simulink model "ASM_Traffic_new"  (R2024a)
settings: Solver=ode1  StartTime=SIM.tstart.v  StopTime=SIM.tend.v  FixedStep=SIM.StepSize.v  RelTol=1e-3
PostLoadFcn:
  | if any(exist('dsrtsu_mdlpostloadfcn', 'file') ~= 0), dsrtsu_mdlpostloadfcn('Execute', bdroot); end
  | try, asm_mdl_postloadfcn(bdroot, 'UpdateModel', 3600); catch, disp(lasterr); end,
InitFcn:
  | , if any(exist('rtifpga_mdlclblib', 'file') ~= 0), rtifpga_mdlclblib('Init', bdroot); end,
  | , if any(exist('dsmpb_private', 'file') ~= 0), dsmpb_private('dsmpb_mdlclblib', 'Init', bdroot); end,
undefined symbols (not defined in the file): _to_, a0b2, ASM_BrakeHydraulics_DemoSystems, ASM_VehicleDynamics_DemoSystems, b98103fe8ad365046cd0, BrakeCircuit, CPT, Crankshaft, DiscIntNeverNeededParam, dsmsi, FinalDriveAssembly, MDL, ModeSignals, Pos_BrakePedal_Maneuver, rad, RefSignals, s_to_rpm, SIM, SoftECU, Suspension, Tire, Transmission
libraries: ASM_Traffic_lib x135, simulink x100, ASM_Utils_lib x77, ASM_VehicleDynamics_lib x70, ASM_Environment_lib x22, dsmpblib x20, dsmsilib x15, MDLD_Utils_lib x10, ASM_BrakeHydraulics_lib x3
(part 32 of 63)

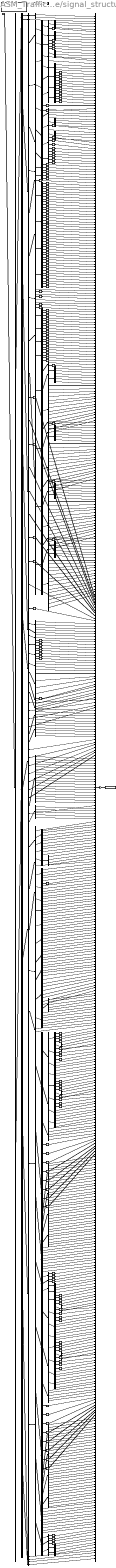
== system ASM_Traffic_new/VehicleDynamics/SignalInterface/ASMSignalInterface/signal_structure ==
  ASMSignalBus : Inport
  Accelerations : BusSelector  OutputSignals=VehicleCoG,Wheels
  ActiveBrakeCylinder : BusSelector  OutputSignals=p[bar],p_max[bar],Enable_p_Brake_Desired[0|1],p_Brake_Desired[bar]
  Aerodynamics : BusSelector  OutputSignals=Forces,Torques,Coefficients
  Angle_FL_Wheel[Toe;Camber][deg] : BusSelector  OutputSignals=Angle_Toe_FL_Wheel_CoorSys_V[deg],Angle_Camber_FL_Wheel_CoorSys_V[deg]
  Angle_FR_Wheel[Toe;Camber][deg] : BusSelector  OutputSignals=Angle_Toe_FR_Wheel_CoorSys_V[deg],Angle_Camber_FR_Wheel_CoorSys_V[deg]
  Angle_Left_Wheel[Alpha;Beta;Gamma][deg] : BusSelector  OutputSignals=Angle_Alpha_Left_Wheel[deg],Angle_Beta_Left_Wheel[deg],Angle_Gamma_Left_Wheel[deg]
  Angle_Left_Wheel[Alpha;Beta;Gamma][deg]1 : BusSelector  OutputSignals=Angle_Alpha_Left_Wheel[deg],Angle_Beta_Left_Wheel[deg],Angle_Gamma_Left_Wheel[deg]
  Angle_RL_Wheel[Toe;Camber][deg] : BusSelector  OutputSignals=Angle_Toe_RL_Wheel_CoorSys_V[deg],Angle_Camber_RL_Wheel_CoorSys_V[deg]
  Angle_RR_Wheel[Toe;Camber][deg] : BusSelector  OutputSignals=Angle_Toe_RR_Wheel_CoorSys_V[deg],Angle_Camber_RR_Wheel_CoorSys_V[deg]
  Angle_Right_Wheel[Alpha;Beta;Gamma][deg] : BusSelector  OutputSignals=Angle_Alpha_Right_Wheel[deg],Angle_Beta_Right_Wheel[deg],Angle_Gamma_Right_Wheel[deg]
  Angle_Right_Wheel[Alpha;Beta;Gamma][deg]1 : BusSelector  OutputSignals=Angle_Alpha_Right_Wheel[deg],Angle_Beta_Right_Wheel[deg],Angle_Gamma_Right_Wheel[deg]
  Angle_Vehicle_CoorSys_E[x;y;z][deg] : BusSelector  OutputSignals=Angle_Roll_Vehicle_CoorSys_E[deg],Angle_Pitch_Vehicle_CoorSys_E[deg],Angle_Yaw_Vehicle_CoorSys_E[deg]
  Angle_Wheel[FL;FR][Toe;Camber][deg] : BusSelector  OutputSignals=Angle_FL_Wheel[Toe;Camber][deg],Angle_FR_Wheel[Toe;Camber][deg]
  Angle_Wheel[RL;RR][Toe;Camber][deg] : BusSelector  OutputSignals=Angle_RL_Wheel[Toe;Camber][deg],Angle_RR_Wheel[Toe;Camber][deg]
  Angular : BusSelector  OutputSignals=w_Vehicle_CoG_dt[x;y;z][rad|s2]
  Angular1 : BusSelector  OutputSignals=w_Vehicle_CoG[x;y;z][deg|s]
  Angular2 : BusSelector  OutputSignals=WheelBodyAngularVelocity,WheelAngularVelocity
  Angular3 : BusSelector  OutputSignals=Angle_Vehicle_CoorSys_E[x;y;z][deg],Angle_V[Alpha;Beta;Gamma][deg],RotationMatrix_V_to_E[3x3],RotationMatrix_V_to_E[1x9],RotationMatrix_V_to_E_T[3x3],RotationMatrix_V_to_E_T[1x9]
  BellValve : BusSelector  OutputSignals=ValveState[1ChamberCon|2AmbientCon|3CloseAll],p_In_BellValve[bar],p_Out_BellValve[bar],T_In_BellValve[degC],m_dot_BellValve[kg|s],Ctrl_BellValve[0_1]
  Brake : BusSelector  OutputSignals=MasterBrakeCylinder,BrakeHydraulics,BrakeDisc,VacuumServo,Manifold
  BrakeCylinderLinear : BusSelector  OutputSignals=p[bar],p_max[bar]
  BrakeCylinderPhysical : BusSelector  OutputSignals=Displ_Piston[mm],F[N],p[bar],p_max[bar]
  BrakeDisc : BusSelector  OutputSignals=Torque,MaximumTorque,Pressure,Const_BrakeDiscFactor
  BrakeHydraulics : BusSelector  OutputSignals=BrakingCircuit,BrakeHydraulicsModel[]
  BrakingCircuit : BusSelector  OutputSignals=Pressure
  BusSelector_1 : BusSelector  OutputSignals=Control,Plant
  Coefficients : BusSelector  OutputSignals=Cw_x[]
  ComplianceAligningTorque : BusSelector  OutputSignals=Displ_x_Wheel_Trq_z_Left[mm],Displ_x_Wheel_Trq_z_Right[mm],Displ_y_Wheel_Trq_z_Left[mm],Displ_y_Wheel_Trq_z_Right[mm],Angle_Alpha_Wheel_Trq_z_Left[deg],Angle_Alpha_Wheel_Trq_z_Right[deg],Angle_Gamma_Wheel_Trq_z_Left[deg],Angle_Gamma_Wheel_Trq_z_Right[deg]
  ComplianceAligningTorque1 : BusSelector  OutputSignals=Displ_x_Wheel_Trq_z_Left[mm],Displ_x_Wheel_Trq_z_Right[mm],Displ_y_Wheel_Trq_z_Left[mm],Displ_y_Wheel_Trq_z_Right[mm],Angle_Alpha_Wheel_Trq_z_Left[deg],Angle_Alpha_Wheel_Trq_z_Right[deg],Angle_Gamma_Wheel_Trq_z_Left[deg],Angle_Gamma_Wheel_Trq_z_Right[deg]
  ComplianceLatForce : BusSelector  OutputSignals=Displ_x_Wheel_F_y_Left[mm],Displ_x_Wheel_F_y_Right[mm],Displ_y_Wheel_F_y_Left[mm],Displ_y_Wheel_F_y_Right[mm],Angle_Alpha_Wheel_F_y_Left[deg],Angle_Alpha_Wheel_F_y_Right[deg],Angle_Gamma_Wheel_F_y_Left[deg],Angle_Gamma_Wheel_F_y_Right[deg]
  ComplianceLatForce1 : BusSelector  OutputSignals=Displ_x_Wheel_F_y_Left[mm],Displ_x_Wheel_F_y_Right[mm],Displ_y_Wheel_F_y_Left[mm],Displ_y_Wheel_F_y_Right[mm],Angle_Alpha_Wheel_F_y_Left[deg],Angle_Alpha_Wheel_F_y_Right[deg],Angle_Gamma_Wheel_F_y_Left[deg],Angle_Gamma_Wheel_F_y_Right[deg]
  ComplianceLongForce : BusSelector  OutputSignals=Displ_x_Wheel_F_x_Left[mm],Displ_x_Wheel_F_x_Right[mm],Displ_y_Wheel_F_x_Left[mm],Displ_y_Wheel_F_x_Right[mm],Angle_Alpha_Wheel_F_x_Left[deg],Angle_Alpha_Wheel_F_x_Right[deg],Angle_Gamma_Wheel_F_x_Left[deg],Angle_Gamma_Wheel_F_x_Right[deg]
  ComplianceLongForce1 : BusSelector  OutputSignals=Displ_x_Wheel_F_x_Left[mm],Displ_x_Wheel_F_x_Right[mm],Displ_y_Wheel_F_x_Left[mm],Displ_y_Wheel_F_x_Right[mm],Angle_Alpha_Wheel_F_x_Left[deg],Angle_Alpha_Wheel_F_x_Right[deg],Angle_Gamma_Wheel_F_x_Left[deg],Angle_Gamma_Wheel_F_x_Right[deg]
  ComplianceLongTorque : BusSelector  OutputSignals=Displ_x_Wheel_Trq_x_Left[mm],Displ_x_Wheel_Trq_x_Right[mm],Displ_y_Wheel_Trq_x_Left[mm],Displ_y_Wheel_Trq_x_Right[mm],Angle_Alpha_Wheel_Trq_x_Left[deg],Angle_Alpha_Wheel_Trq_x_Right[deg],Angle_Gamma_Wheel_Trq_x_Left[deg],Angle_Gamma_Wheel_Trq_x_Right[deg]
  ComplianceLongTorque1 : BusSelector  OutputSignals=Displ_x_Wheel_Trq_x_Left[mm],Displ_x_Wheel_Trq_x_Right[mm],Displ_y_Wheel_Trq_x_Left[mm],Displ_y_Wheel_Trq_x_Right[mm],Angle_Alpha_Wheel_Trq_x_Left[deg],Angle_Alpha_Wheel_Trq_x_Right[deg],Angle_Gamma_Wheel_Trq_x_Left[deg],Angle_Gamma_Wheel_Trq_x_Right[deg]
  Const_BrakeDiscFactor : BusSelector  OutputSignals=Const_BrakeDiscFactor_FL[m3],Const_BrakeDiscFactor_FR[m3],Const_BrakeDiscFactor_RL[m3],Const_BrakeDiscFactor_RR[m3]
  ContactPoint{,1..3} (4 alike) : BusSelector  OutputSignals=r_Tire[m],Pos_CP_CoorSys_E[x;y][m]
  ContentID : Constant  Value=957506836
  Control : BusSelector  OutputSignals=SoftECU_Brake,SoftECU_PowerSteering
  ControllerBellValve : BusSelector  OutputSignals=p_Setpoint[bar],p_MasterBrakeCyl[bar],p_delta[bar],ValveState[1ChamberCon|2AmbientCon],Ctrl_A_BellValve[0_1],F_Pedal[N]
  Damper_Left : BusSelector  OutputSignals=Displ_Damper_Left_dt[m|s],Displ_Damper_Left_dqL[],Displ_Damper_Left_dqR[],Displ_Damper_Left[m]
  Damper_Left1 : BusSelector  OutputSignals=Displ_Damper_Left_dt[m|s],Displ_Damper_Left_dqL[],Displ_Damper_Left_dqR[],Displ_Damper_Left[m]
  Damper_Right : BusSelector  OutputSignals=Displ_Damper_Right_dt[m|s],Displ_Damper_Right_dqL[],Displ_Damper_Right_dqR[],Displ_Damper_Right[m]
  Damper_Right1 : BusSelector  OutputSignals=Displ_Damper_Right_dt[m|s],Displ_Damper_Right_dqL[],Displ_Damper_Right_dqR[],Displ_Damper_Right[m]
  DesiredBrakePressure : BusSelector  OutputSignals=Enable_p_Brake_Desired[0|1],p_Brake_Desired[bar]
  DrivingResistances : BusSelector  OutputSignals=F_Driving_Res[N]
  F_Tire_CoorSys_V[x;y;z][N]{,1..3} (4 alike) : BusSelector  OutputSignals=F_x_Tire_CoorSys_V[N],F_y_Tire_CoorSys_V[N],F_z_Tire_CoorSys_V[N]
  Forces : BusSelector  OutputSignals=F_x_Aero_CoorSys_V[N],F_y_Aero_CoorSys_V[N],F_z_Aero_CoorSys_V[N]
  ForcesAndTorques : BusSelector  OutputSignals=g_F_Steering_SteeringRod[N],Trq_Steering[Nm],Trq_PowerSteering[Nm],TrqSpring_SteeringColumn[Nm],Trq_PowerSteeringDynamics[Nm],TrqSpring_PowerSteeringSystem[Nm]
  Generalized : BusSelector  OutputSignals=v_Vehicle[x;y;z][km|h],w_Vehicle[x;y;z][deg|s],z_Wheel_dt[FL;FR;RL;RR][m|s]
  GeneralizedForcesAndTorques : BusSelector  OutputSignals=g_F_Vehicle[x;y;z][N],g_Trq_Vehicle[x;y;z][Nm],g_F_z_Wheel[FL;FR;RL;RR][N]
  GeneralizedForcesAndTorques1 : BusSelector  OutputSignals=g_FTrq_Tire_Steering[N],g_Trq_FL_Steering[N],g_Trq_FR_Steering[N],g_F_FL_Steering[N],g_F_FR_Steering[N]
  GeneralizedVelocitiesDerivative : BusSelector  OutputSignals=v_Vehicle_dt[x;y;z][m|s2],w_Vehicle_dt[x;y;z][rad|s2],q_Wheel_dt2[q1_Front;q2_Front;q1_Rear;q2_Rear][]
  GravitationalForces : BusSelector  OutputSignals=F_Vehicle_Gravitational[x;y;z][N],F_FL_Gravitational[x;y;z][N],F_FR_Gravitational[x;y;z][N],F_RL_Gravitational[x;y;z][N],F_RR_Gravitational[x;y;z][N]
  GravityAcceleration : BusSelector  OutputSignals=a_Gravity_CoorSys_V[x;y;z][m|s2]
  GyroscopicForces : BusSelector  OutputSignals=F_Vehicle_Gyroscopic[x;y;z][N],F_FL_Gyroscopic[x;y;z][N],F_FR_Gyroscopic[x;y;z][N],F_RL_Gyroscopic[x;y;z][N],F_RR_Gyroscopic[x;y;z][N]
  GyroscopicTorques : BusSelector  OutputSignals=Trq_Vehicle_Gyroscope[x;y;z][Nm],Trq_FL_Gyroscope[x;y;z][Nm],Trq_FR_Gyroscope[x;y;z][Nm],Trq_RL_Gyroscope[x;y;z][Nm],Trq_RR_Gyroscope[x;y;z][Nm]
  InfoBlock : Subsystem
      mask Display: fprintf('Structural changes of the signal bus require an update \nof the ''ASMSignalCollector'' block. \n\nTo start the update process double click the parent block.\n\n WARNING:\n During update this subsystem will be cleared completely')
  Kinematics_Left : BusSelector  OutputSignals=Position_Left,Orientation_Left,Spring_Left,Damper_Left
  Kinematics_Left1 : BusSelector  OutputSignals=Position_Left,Orientation_Left,Spring_Left,Damper_Left
  Kinematics_Right : BusSelector  OutputSignals=Position_Right,Orientation_Right,Spring_Right,Damper_Right
  Kinematics_Right1 : BusSelector  OutputSignals=Position_Right,Orientation_Right,Spring_Right,Damper_Right
  Linear : BusSelector  OutputSignals=a_Vehicle_CoG[x;y;z][m|s2],a_Vehicle_CoG_withG[x;y;z][m|s2]
  Linear1 : BusSelector  OutputSignals=a_FL_Wheel[x;y;z][m|s2],a_FR_Wheel[x;y;z][m|s2],a_RL_Wheel[x;y;z][m|s2],a_RR_Wheel[x;y;z][m|s2]
  Linear2 : BusSelector  OutputSignals=v_Vehicle_CoG[x;y;z][km|h],v_Total_Vehicle[km|h],Angle_SideSlip_Vehicle[deg]
  Linear3 : BusSelector  OutputSignals=WheelBodyVelocity
  Linear4 : BusSelector  OutputSignals=Pos_Vehicle_CoorSys_E[x;y;z][m],Pos_Vehicle_CoorSys_E[m],s_Vehicle[m]
  Linear5 : BusSelector  OutputSignals=Pos_FL_Wheels_CoorSys_E[x;y;z][m],Pos_FR_Wheels_CoorSys_E[x;y;z][m],Pos_RL_Wheels_CoorSys_E[x;y;z][m],Pos_RR_Wheels_CoorSys_E[x;y;z][m]
  MDLD_DATA_CAPTURE : MDLD_Utils_lib/ModelDeskPlotInterface/DataCapture_Sfcn/MDLD_DATA_CAPTURE  inputPortWidth=976  measurementSignals=[0 0 0 0 0 0 0 0 0 0 0 0 0 0 0 0 0 0 0 0 0 0 0 0 0 0 0 0 0 0 0 0 0 0 0 0 0 0 0 0 0 0 0 0 0 0 0 0 0 0 0 0 0 0 0 0 0 0 0 0 0 0 0 0 0 0 0 0 0 0 0 0 0 0 0 0 0 0 0 0 0 0 0 0 0 0 0 0 0 0 0 0 0 0 0 0 0 0 0 0 0 0 0 0 0 0 0 0 0 0 0 0 0 0 0 0 0 0 0 0 0 0 0 0 0 0 0 0 0 0 0 0 0 0 0 0 0 0 0 0 0 0 0 0 0 0 0 0 0 0 0 0 0 0 0 0 0 0 0 0 0 0 0 0 0 0 0 0 0 0 0 0 0 0 0 0 0 0 0 0 0 0 0 0 0 0 0 0 0 0 0 0 0 0 0 0 0 0 0 0 0 0 0 0 0 0 0 0 0 0 0 0 0 0 0 0 0 0 0 0 0 0 0 0 0 0 0 0 0 0 0 0 0 0 0 0 0 0 0 0 0 0 0 0 0 0 0 0 0 0 0 0 0 0 0 0 0 0 0 0 0 0 0 0 0 0 0 0 0 0 0 0 0 0 0 0 0 0 0 0 0 0 0 0 0 0 0 0 0 0 0 0 0 0 0 0 0 0 0 0 0 0 0 0 0 0 0 0 0 0 0 0 0 0 0 0 0 0 0 0 0 0 0 0 0 0 0 0 0 0 0 0 0 0 0 0 0 0 0 0 0 0 0 0 0 0 0 0 0 0 0 0 0 0 0 0 0 0 0 0 0 0 0 0 0 0 0 0 0 0 0 0 0 0 0 0 0 0 0 0 0 0 0 0 0 0 0 0 0 0 0 0 0 0 0 0 0 0 0 0 0 0 0 0 0 0 0 0 0 0 0 0 0 0 0 0 0 0 0 0 0 0 0 0 0 0 0 0 0 0 0 0 0 0 0 0 0 0 0 0 0 0 0 0 0 0 0 0 0 0 0 0 0 0 0 0 0 0 0 0 0 0 0 0 0 0 0 0 0 0 0 0 0 0 0 0 0 0 0 0 0 0 0 0 0 0 0 0 0 0 0 0 0 0 0 0 0 0 0 0 0 0 0 0 0 0 0 0 0 0 0 0 0 0 0 0 0 0 0 0 0 0 0 0 0 0 0 0 0 0 0 0 0 0 0 0 0 0 0 0 0 0 0 0 0 0 0 0 0 0 0 0 0 0 0 0 0 0 0 0 0 0 0 0 0 0 0 0 0 0 0 0 0 0 0 0 0 0 0 0 0 0 0 0 0 0 0 0 0 0 0 0 0 0 0 0 0 0 0 0 0 0 0 0 0 0 0 0 0 0 0 0 0 0 0 0 0 0 0 0 0 0 0 0 0 0 0 0 0 0 0 0 0 0 0 0 0 0 0 0 0 0 0 0 0 0 0 0 0 0 0 0 0 0 0 0 0 0 0 0 0 0 0 0 0 0 0 0 0 0 0 0 0 0 0 0 0 0 0 0 0 0 0 0 0 0 0 0 0 0 0 0 0 0 0 0 0 0 0 0 0 0 0 0 0 0 0 0 0 0 0 0 0 0 0 0 0 0 0 0 0 0 0 0 0 0 0 0 0 0 0 0 0 0 0 0 0 0 0 0 0 0 0 0 0 0 0 0 0 0 0 0 0 0 0 0 0 0 0 0 0 0 0 0 0 0 0 0 0 0 0 0 0 0 0 0 0 0 0 0 0 0 0 0 0 0 0 0 0 0 0 0 0 0 0 0 0 0 0 0 0 0 0 0 0 0 0 0 0 0 0 0 0 0 0 0 0 0 0 0 0 0 0 0 0 0 0 0 0 0 0 0 0 0 0 0 0 0 0 0 0 0 0 0 0 0 0 0 0 0 0 0 0 0 0 0 0 0 0 0 0 0 0 0 0 0 0 0 0 0 0 0 0 0 0 0 0 0 0 0 0 0 0 0 0 0 0 0 0 0 0 0 0 0 0 0 0 0 0 0 0 0 0 0 0 0 0 0 0 0 0 0 0 0 0 0 0 0 0 0 0 0 0 0 0 0 0 0 0 0 0 0 0 0 0 0 0 0 0 0 0 0 0 0 0 0 0 0 0 0 0 0 0 0 0 0 0 0 0 0 0 0 0 0 0 0 0 0 0 0 0 0 0 0 0 0]  downsampling=1  samplingPeriod=SIM.StepSize.v  uuid=0  ASMProperties=struct('Name','mdld_data_capture','Version','1.0','Library','mdld_utils_lib')  startTriggerDelay=0  startTriggerLogic=0  startTriggerCount=0  startTriggerConditions=[0,0,0,0,0,0,0,0,0]  stopTriggerDelay=0  stopTriggerLogic=0  stopTriggerCount=0  stopTriggerConditions=[0,0,0,0,0,0,0,0,0]  ContentID_RefStruct=957506836
  Manifold : BusSelector  OutputSignals=Pos_AccPedal[%],p_Manifold[bar]
  ManifoldValve : BusSelector  OutputSignals=p_In_MainfoldValve[bar],p_Out_MainfoldValve[bar],T_In_MainfoldValve[degC],m_dot_ManifoldValve[kg|s],m_dot_Out_ManifoldValve[kg|s],m_dot_In_ManifoldValve[kg|s]
  MassForcesAndTorques : BusSelector  OutputSignals=GravitationalForces,GyroscopicForces,GyroscopicTorques,ResidualAccelerations
  MasterBrakeCylinder : BusSelector  OutputSignals=Sw_MasterBrakeCylinder_Mode[1linear|2physical|3Booster|4BrakeByWire],ActiveBrakeCylinder,BrakeCylinderLinear,BrakeCylinderPhysical
  MaximumTorque : BusSelector  OutputSignals=Trq_Max_Brake[Nm],Trq_Max_Brake[FL;FR;RL;RR][Nm],Trq_FL_max_Brake[Nm],Trq_FR_max_Brake[Nm],Trq_RL_max_Brake[Nm],Trq_RR_max_Brake[Nm]
  Orientation_Left : BusSelector  OutputSignals=Angle_Left_Wheel[Alpha;Beta;Gamma][deg],w_Rel_Left_Wheel_dqL_dt[x;y;z][rad|m],w_Rel_Left_Wheel_dqR_dt[x;y;z][rad|m],w_Rel_Left_Wheel_dDispl_SteeringRod_dt[x;y;z][rad|m],UnitVec_y_Wheel_Left_CoorSys_V[x;y;z]
  Orientation_Left1 : BusSelector  OutputSignals=Angle_Left_Wheel[Alpha;Beta;Gamma][deg],w_Rel_Left_Wheel_dqL_dt[x;y;z][rad|m],w_Rel_Left_Wheel_dqR_dt[x;y;z][rad|m],w_Rel_Left_Wheel_dDispl_SteeringRod_dt[x;y;z][rad|m],UnitVec_y_Wheel_Left_CoorSys_V[x;y;z]
  Orientation_Right : BusSelector  OutputSignals=Angle_Right_Wheel[Alpha;Beta;Gamma][deg],w_Rel_Right_Wheel_dqL_dt[x;y;z][rad|m],w_Rel_Right_Wheel_dqR_dt[x;y;z][rad|m],w_Rel_Right_Wheel_dDispl_SteeringRod_dt[x;y;z][rad|m],UnitVec_y_Wheel_Right_CoorSys_V[x;y;z]
  Orientation_Right1 : BusSelector  OutputSignals=Angle_Right_Wheel[Alpha;Beta;Gamma][deg],w_Rel_Right_Wheel_dqL_dt[x;y;z][rad|m],w_Rel_Right_Wheel_dqR_dt[x;y;z][rad|m],w_Rel_Right_Wheel_dDispl_SteeringRod_dt[x;y;z][rad|m],UnitVec_y_Wheel_Right_CoorSys_V[x;y;z]
  OutputPoint : BusSelector  OutputSignals=F_OutputPoint[N],p_OutputPoint[bar],Pos_BrakePedal_OutputPoint[%],F_Max_Pedal[N],p_Max_Booster[bar]
  Plant : BusSelector  OutputSignals=VehicleMovement,Tire,Aerodynamics,Wheel,Steering,Brake,Suspension,SteeringRod_Back_Calc,DrivingResistances
  Pos_Vehicle_CoorSys_E[x;y;z][m] : BusSelector  OutputSignals=Pos_x_Vehicle_CoorSys_E[m],Pos_y_Vehicle_CoorSys_E[m],Pos_z_Vehicle_CoorSys_E[m]
  Pos_Wheel[FL;FR][x;y;z][m] : BusSelector  OutputSignals=Pos_FL_Wheel[x;y;z][m],Pos_FR_Wheel[x;y;z][m]
  Pos_Wheel[RL;RR][x;y;z][m] : BusSelector  OutputSignals=Pos_RL_Wheel[x;y;z][m],Pos_RR_Wheel[x;y;z][m]
  Position_Left : BusSelector  OutputSignals=Pos_Left_Wheel[x;y;z][m],Pos_Left_Wheel_dqL[x;y;z][],Pos_Left_Wheel_dqR[x;y;z][],Pos_Left_Wheel_dDispl_SteeringRod[x;y;z][]
  Position_Left1 : BusSelector  OutputSignals=Pos_Left_Wheel[x;y;z][m],Pos_Left_Wheel_dqL[x;y;z][],Pos_Left_Wheel_dqR[x;y;z][],Pos_Left_Wheel_dDispl_SteeringRod[x;y;z][]
  Position_Right : BusSelector  OutputSignals=Pos_Right_Wheel[x;y;z][m],Pos_Right_Wheel_dqL[x;y;z][],Pos_Right_Wheel_dqR[x;y;z][],Pos_Right_Wheel_dDispl_SteeringRod[x;y;z][]
  Position_Right1 : BusSelector  OutputSignals=Pos_Right_Wheel[x;y;z][m],Pos_Right_Wheel_dqL[x;y;z][],Pos_Right_Wheel_dqR[x;y;z][],Pos_Right_Wheel_dDispl_SteeringRod[x;y;z][]
  Positions : BusSelector  OutputSignals=Vehicle,Wheels
  Pressure : BusSelector  OutputSignals=p_FL_Brake[bar],p_FR_Brake[bar],p_RL_Brake[bar],p_RR_Brake[bar]
  Pressure1 : BusSelector  OutputSignals=p_FL_Brake[bar],p_FR_Brake[bar],p_RL_Brake[bar],p_RR_Brake[bar]
  PushRod : BusSelector  OutputSignals=F_Pedal[N],F_Spring[N],F_RearChamber[N],F_VacuumChamber[N],F_PushRod[N],x[m],V_delta[m3],A_Diaphragm[m2],OutputPoint
  RearChamber : BusSelector  OutputSignals=m_dot_In_RearChamber[kg|s],m_dot_Out_RearChamber[kg|s],T_RearChamber[degC],p_RearChamber[bar],V_RearChamber[m3]
  RelativePositionFront : BusSelector  OutputSignals=Pos_Wheel[FL;FR][x;y;z][m],UnitVec_y_Wheel_CoorSys_V[FL;FR][x;y;z],Angle_Wheel[FL;FR][Toe;Camber][deg]
  RelativePositionRear : BusSelector  OutputSignals=Pos_Wheel[RL;RR][x;y;z][m],UnitVec_y_Wheel_CoorSys_V[RL;RR][x;y;z],Angle_Wheel[RL;RR][Toe;Camber][deg]
  Reshape_{7,11..14,23..36,44,49..104,106,108,111..132,134,156,178,200,221,223,227..228,230,238..245,254,327,384..387,391..394,402..405,409..412,425..432,475..478,483..486,490..493,501..504,508..511,524..531,574..577} (175 alike) : Reshape
  ResidualAccelerations : BusSelector  OutputSignals=a_Vehicle_CoG_Residual[x;y;z][m|s2],a_FL_Residual[x;y;z][m|s2],a_FR_Residual[x;y;z][m|s2],a_RL_Residual[x;y;z][m|s2],a_RR_Residual[x;y;z][m|s2]
  RotationAngle : BusSelector  OutputSignals=Angle_Rot_FL_Wheel[deg],Angle_Rot_FR_Wheel[deg],Angle_Rot_RL_Wheel[deg],Angle_Rot_RR_Wheel[deg]
  Sensor1 : BusSelector  OutputSignals=a_Angular_Sensor1_CoorSys_V[x;y;z][rad|s2],a_Total_Sensor1_CoorSys_V[x;y;z][m|s2],a_Sensor1_CoorSys_V[x;y;z][m|s2],v_Sensor1_CoorSys_V[x;y;z][m|s],w_Sensor1_CoorSys_V[x;y;z][rad|s],a_Angular_Sensor1_CoorSys_VH[x;y;z][rad|s2],a_Total_Sensor1_CoorSys_VH[x;y;z][m|s2],a_Sensor1_CoorSys_VH[x;y;z][m|s2],v_Sensor1_CoorSys_VH[x;y;z][m|s],w_Sensor1_CoorSys_VH[x;y;z][rad|s]
  Sensor2 : BusSelector  OutputSignals=a_Angular_Sensor2_CoorSys_V[x;y;z][rad|s2],a_Total_Sensor2_CoorSys_V[x;y;z][m|s2],a_Sensor2_CoorSys_V[x;y;z][m|s2],v_Sensor2_CoorSys_V[x;y;z][m|s],w_Sensor2_CoorSys_V[x;y;z][rad|s],a_Angular_Sensor2_CoorSys_VH[x;y;z][rad|s2],a_Total_Sensor2_CoorSys_VH[x;y;z][m|s2],a_Sensor2_CoorSys_VH[x;y;z][m|s2],v_Sensor2_CoorSys_VH[x;y;z][m|s],w_Sensor2_CoorSys_VH[x;y;z][rad|s]
  Sensor3 : BusSelector  OutputSignals=a_Angular_Sensor3_CoorSys_V[x;y;z][rad|s2],a_Total_Sensor3_CoorSys_V[x;y;z][m|s2],a_Sensor3_CoorSys_V[x;y;z][m|s2],v_Sensor3_CoorSys_V[x;y;z][m|s],w_Sensor3_CoorSys_V[x;y;z][rad|s],a_Angular_Sensor3_CoorSys_VH[x;y;z][rad|s2],a_Total_Sensor3_CoorSys_VH[x;y;z][m|s2],a_Sensor3_CoorSys_VH[x;y;z][m|s2],v_Sensor3_CoorSys_VH[x;y;z][m|s],w_Sensor3_CoorSys_VH[x;y;z][rad|s]
  Sensor4 : BusSelector  OutputSignals=a_Angular_Sensor4_CoorSys_V[x;y;z][rad|s2],a_Total_Sensor4_CoorSys_V[x;y;z][m|s2],a_Sensor4_CoorSys_V[x;y;z][m|s2],v_Sensor4_CoorSys_V[x;y;z][m|s],w_Sensor4_CoorSys_V[x;y;z][rad|s],a_Angular_Sensor4_CoorSys_VH[x;y;z][rad|s2],a_Total_Sensor4_CoorSys_VH[x;y;z][m|s2],a_Sensor4_CoorSys_VH[x;y;z][m|s2],v_Sensor4_CoorSys_VH[x;y;z][m|s],w_Sensor4_CoorSys_VH[x;y;z][rad|s]
  SensorMotion : BusSelector  OutputSignals=Sensor1,Sensor2,Sensor3,Sensor4
  ShaftsTorques_CoorSys_V : BusSelector  OutputSignals=Trq_Shaft_FL_CoorSys_V[x;y;z][Nm],Trq_Shaft_FR_CoorSys_V[x;y;z][Nm],Trq_Shaft_RL_CoorSys_V[x;y;z][Nm],Trq_Shaft_RR_CoorSys_V[x;y;z][Nm]
  SignalFilter : Mux  Inputs=585
  SignalFilterGain : Gain
  SoftECU_Brake : BusSelector  OutputSignals=DesiredBrakePressure
  SoftECU_PowerSteering : BusSelector  OutputSignals=Trq_PowerSteering[Nm]
  Spring_Left : BusSelector  OutputSignals=Displ_Spring_Left[m],Displ_Spring_Left_dqL[],Displ_Spring_Left_dqR[]
  Spring_Left1 : BusSelector  OutputSignals=Displ_Spring_Left[m],Displ_Spring_Left_dqL[],Displ_Spring_Left_dqR[]
  Spring_Right : BusSelector  OutputSignals=Displ_Spring_Right[m],Displ_Spring_Right_dqL[],Displ_Spring_Right_dqR[]
  Spring_Right1 : BusSelector  OutputSignals=Displ_Spring_Right[m],Displ_Spring_Right_dqL[],Displ_Spring_Right_dqR[]
  Stabilizer : BusSelector  OutputSignals=Displ_Stabilizer[m],Displ_Stabilizer_Left[m],Displ_Stabilizer_Right[m],Displ_Stabilizer_dqL[],Displ_Stabilizer_dqR[]
  Stabilizer1 : BusSelector  OutputSignals=Displ_Stabilizer[m],Displ_Stabilizer_Left[m],Displ_Stabilizer_Right[m],Displ_Stabilizer_dqL[],Displ_Stabilizer_dqR[]
  StatesSteeringSystem : BusSelector  OutputSignals=Angle_EPSSystem[deg],Angle_EPSSystem_dt[deg|s],Angle_LowerSteeringColumn[deg],Angle_LowerSteeringColumn_dt[deg|s],Angle_UpperSteeringColumn[deg],Angle_UpperSteeringColumn_dt[deg|s],Angle_SteeringWheel[deg],Angle_SteeringWheel_dt[deg|s],Displ_Steering[m],Displ_Steering_dt[m|s],Displ_SteeringRod_dt2[m|s2],Angle_SteeringGear[deg],Angle_SteeringGear_dt[deg|s],Angle_EPSPinion[rad],Angle_EPSPinion_dt[rad|s],i_Steering[rad|m],FrictionForce_SteeringRod[N],i_Steering_Wheel2Rod[rad|m]
  Steering : BusSelector  OutputSignals=Displ_Steering[m],Displ_Steering_dt[m|s],Displ_SteeringRod_dt2[m|s2],m_Steering[kg],ForcesAndTorques,GeneralizedForcesAndTorques,i_Steering[rad|m],i_Steering_Mean[],Angle_SteeringGear[deg],Angle_SteeringWheel[deg],Angle_SteeringGear_dt[deg|s],Angle_SteeringWheel_dt[deg|s],Const_Stiffness_SteeringColumn[Nm|rad],StatesSteeringSystem,FrictionTrq_SteeringSystem[Nm],SteeringWheelTorque
  SteeringRod_Back_Calc : BusSelector  OutputSignals=Sw_Backward_SteeringRod_Calc[0Off|1On],Displ_SteeringRod[m],Displ_SteeringRod_dt[m|s]
  SteeringWheelTorque : BusSelector  OutputSignals=TrqSensor_Steering[Nm],Trq_Driver[Nm],g_Trq_SteeringWheel[Nm],TrqFriction_SteeringWheel[Nm],Trq_SteeringWheel[Nm]
  Suspension : BusSelector  OutputSignals=SuspensionFront,SuspensionRear
  SuspensionComplianceFront : BusSelector  OutputSignals=Angle_Comp_FR_Wheel_dt[x;y;z][rad|s],Angle_Comp_FL_Wheel_dt[x;y;z][rad|s],Angle_Comp_FR_Wheel[x;y;z][rad],Angle_Comp_FL_Wheel[x;y;z][rad],Displ_Comp_FR_Wheel_dt[x;y;z][m|s],Displ_Comp_FL_Wheel_dt[x;y;z][m|s],Displ_Comp_FR_Wheel[x;y;z][m],Displ_Comp_FL_Wheel[x;y;z][m],ComplianceLongForce,ComplianceLatForce,ComplianceAligningTorque,ComplianceLongTorque
  SuspensionComplianceRear : BusSelector  OutputSignals=Angle_Comp_RR_Wheel_dt[x;y;z][rad|s],Angle_Comp_RL_Wheel_dt[x;y;z][rad|s],Angle_Comp_RR_Wheel[x;y;z][rad],Angle_Comp_RL_Wheel[x;y;z][rad],Displ_Comp_RR_Wheel_dt[x;y;z][m|s],Displ_Comp_RL_Wheel_dt[x;y;z][m|s],Displ_Comp_RR_Wheel[x;y;z][m],Displ_Comp_RL_Wheel[x;y;z][m],ComplianceLongForce,ComplianceLatForce,ComplianceAligningTorque,ComplianceLongTorque
  SuspensionForcesFront : BusSelector  OutputSignals=F_FL_Spring[N],F_FL_Spring_dDispl_FL_Spring[N|m],F_FL_Damper[N],F_FL_Damper_dDispl_FL_Damper_dt[N|(m|s)],F_Stabilizer[N],F_Stabilizer_dDispl_Stabilizer[N|m],F_FR_Spring[N],F_FR_Spring_dDispl_FR_Spring[N|m],F_FR_Damper[N],F_FR_Damper_dDispl_FR_Damper_dt[N|(m|s)]
  SuspensionForcesRear : BusSelector  OutputSignals=F_RL_Spring[N],F_RL_Spring_dDispl_RL_Spring[N|m],F_RL_Damper[N],F_RL_Damper_dDispl_RL_Damper_dt[N|(m|s)],F_Stabilizer[N],F_Stabilizer_dDispl_Stabilizer[N|m],F_RR_Spring[N],F_RR_Spring_dDispl_RR_Spring[N|m],F_RR_Damper[N],F_RR_Damper_dDispl_RR_Damper_dt[N|(m|s)]
  SuspensionFront : BusSelector  OutputSignals=SuspensionKinematicsFront,SuspensionComplianceFront,SuspensionForcesFront,RelativePositionFront
  SuspensionKinematicsFront : BusSelector  OutputSignals=Kinematics_Left,Kinematics_Right,Stabilizer
  SuspensionKinematicsRear : BusSelector  OutputSignals=Kinematics_Left,Kinematics_Right,Stabilizer
  SuspensionRear : BusSelector  OutputSignals=SuspensionKinematicsRear,SuspensionComplianceRear,SuspensionForcesRear,RelativePositionRear
  Terminator : Terminator
  Tire : BusSelector  OutputSignals=Tire_allSignals,r_Dyn_Tire[FL;FR;RL;RR][m],r_Dyn_Tire_Mean[m],Coef_RollingRes[FL;FR;RL;RR][],Coef_RollingRes_Mean[],CorneringStiffness_Tire_Front[N|rad],CorneringStiffness_Tire_Rear[N|rad],CorneringStiffness[FL;FR;RL;RR][N|rad],Const_r_unloaded_Tire[FL;FR;RL;RR][m],Const_r_unloaded_Tire_Mean[m],Slip_x_Wheel[]
  Tire{1..4} (4 alike) : BusSelector  OutputSignals=v_Circumf_Dyn_Wheel[km|h],Slip_x[],Slip_y[],r_Dyn_Tire[m],CorneringStiffness[N|rad],Coef_RollingRes[],Trq_x_CoorSys_CP[Nm],Trq_y_CoorSys_W[Nm],Trq_z_CoorSys_CP[Nm],F_x_Dyn_Tire_CoorSys_CP[N],F_y_Dyn_Tire_CoorSys_CP[N],F_z_Dyn_Tire_CoorSys_CP[N],Const_r_unloaded_Tire[m],Const_Stiffness_z_Tire[N|m]
  TireForcesAndTorques{,1..3} (4 alike) : BusSelector  OutputSignals=F_Tire_CoorSys_V[x;y;z][N],Trq_Tire_CoorSys_V[x;y;z][Nm]
  TireWheelTorques : BusSelector  OutputSignals=Trq_Tire_Wheel_FL[Nm],Trq_Tire_Wheel_FR[Nm],Trq_Tire_Wheel_RL[Nm],Trq_Tire_Wheel_RR[Nm]
  Tire_FL : BusSelector  OutputSignals=ContactPoint,TireForcesAndTorques,Tire
  Tire_FR : BusSelector  OutputSignals=ContactPoint,TireForcesAndTorques,Tire
  Tire_RL : BusSelector  OutputSignals=ContactPoint,TireForcesAndTorques,Tire
  Tire_RR : BusSelector  OutputSignals=ContactPoint,TireForcesAndTorques,Tire
  Tire_allSignals : BusSelector  OutputSignals=Tire_FL,Tire_FR,Tire_RL,Tire_RR
  Torque : BusSelector  OutputSignals=Trq_FL_Brake[Nm],Trq_FR_Brake[Nm],Trq_RL_Brake[Nm],Trq_RR_Brake[Nm]
  Torques : BusSelector  OutputSignals=Trq_x_Aero_CoorSys_V[Nm],Trq_y_Aero_CoorSys_V[Nm],Trq_z_Aero_CoorSys_V[Nm]
  Trq_Tire_CoorSys_V[x;y;z][Nm]{,1..3} (4 alike) : BusSelector  OutputSignals=Trq_x_Tire_CoorSys_V[Nm],Trq_y_Tire_CoorSys_V[Nm],Trq_z_Tire_CoorSys_V[Nm]
  UnitVec_y_Wheel_CoorSys_V[FL;FR][x;y;z] : BusSelector  OutputSignals=UnitVec_y_FL_Wheel_CoorSys_V[x;y;z],UnitVec_y_FR_Wheel_CoorSys_V[x;y;z]
  UnitVec_y_Wheel_CoorSys_V[RL;RR][x;y;z] : BusSelector  OutputSignals=UnitVec_y_RL_Wheel_CoorSys_V[x;y;z],UnitVec_y_RR_Wheel_CoorSys_V[x;y;z]
  VacuumChamber : BusSelector  OutputSignals=m_dot_In_1_VacuumChamber[kg|s],m_dot_In_2_VacuumChamber[kg|s],m_dot_Out_2_VacuumChamber[kg|s],T_VacuumChamber[degC],p_VacuumChamber[bar],V_VacuumChamber[m3]
  VacuumServo : BusSelector  OutputSignals=ManifoldValve,VacuumChamber,BellValve,RearChamber,PushRod,ControllerBellValve
  Vehicle : BusSelector  OutputSignals=Linear,Angular
  Vehicle1 : BusSelector  OutputSignals=Linear,Angular
  VehicleCoG : BusSelector  OutputSignals=Linear,Angular
  VehicleEquationOfMotion : BusSelector  OutputSignals=GeneralizedForcesAndTorques,GeneralizedVelocitiesDerivative
  VehicleMassAndAdditionalLoads : BusSelector  OutputSignals=m_TotalVehicle[kg],PosVec_CoG_TotalVehicle[x;y;z][m],Pos_x_CoG_Vehicle_Total[m],Inertia_Tensor_TotalVehicle[3x3][kgm2],Inertia_z_Vehicle_Total[kgm2],m_TotalV1[kg],PosVec_CoG_TotalV1[x;y;z][m],Inertia_Tensor_TotalV1[3x3][kgm2]
  VehicleMovement : BusSelector  OutputSignals=Accelerations,Velocities,Positions,VehicleEquationOfMotion,GravityAcceleration,SensorMotion,VehicleMassAndAdditionalLoads,MassForcesAndTorques
  Velocities : BusSelector  OutputSignals=Vehicle,Wheels,Generalized
  Wheel : BusSelector  OutputSignals=WheelSpeed_CoorSys_V,ShaftsTorques_CoorSys_V,TireWheelTorques,WheelSpeed,WheelSpeed2,RotationAngle
  WheelAngularVelocity : BusSelector  OutputSignals=w_FL_Abs_Wheel[x;y;z][rad|s],w_FR_Abs_Wheel[x;y;z][rad|s],w_RL_Abs_Wheel[x;y;z][rad|s],w_RR_Abs_Wheel[x;y;z][rad|s]
  WheelBodyAngularVelocity : BusSelector  OutputSignals=w_FL_Abs_WheelBody[x;y;z][rad|s],w_FR_Abs_WheelBody[x;y;z][rad|s],w_RL_Abs_WheelBody[x;y;z][rad|s],w_RR_Abs_WheelBody[x;y;z][rad|s]
  WheelBodyVelocity : BusSelector  OutputSignals=v_FL_Abs_WheelBody[x;y;z][km|h],v_FR_Abs_WheelBody[x;y;z][km|h],v_RL_Abs_WheelBody[x;y;z][km|h],v_RR_Abs_WheelBody[x;y;z][km|h]
  WheelSpeed : BusSelector  OutputSignals=omega_FL_Wheel[rad|s],omega_FR_Wheel[rad|s],omega_RL_Wheel[rad|s],omega_RR_Wheel[rad|s]
  WheelSpeed2 : BusSelector  OutputSignals=omega_Wheel[FL;FR;RL;RR][rad|s],omega_Mean_Wheel[rad|s]
  WheelSpeed_CoorSys_V : BusSelector  OutputSignals=w_Wheel_FL_CoorSys_V[x;y;z][rad|s],w_Wheel_FR_CoorSys_V[x;y;z][rad|s],w_Wheel_RL_CoorSys_V[x;y;z][rad|s],w_Wheel_RR_CoorSys_V[x;y;z][rad|s]
  Wheels : BusSelector  OutputSignals=Linear
  Wheels1 : BusSelector  OutputSignals=Linear,Angular
  Wheels2 : BusSelector  OutputSignals=Linear
  a_Vehicle_CoG[x;y;z][m|s2] : BusSelector  OutputSignals=a_x_Vehicle_CoG[m|s2],a_y_Vehicle_CoG[m|s2],a_z_Vehicle_CoG[m|s2]
  v_Vehicle_CoG[x;y;z][km|h] : BusSelector  OutputSignals=v_x_Vehicle_CoG[km|h],v_y_Vehicle_CoG[km|h],v_z_Vehicle_CoG[km|h]
  w_Vehicle_CoG[x;y;z][deg|s] : BusSelector  OutputSignals=RollRate_Vehicle_CoG[deg|s],PitchRate_Vehicle_CoG[deg|s],YawRate_Vehicle_CoG[deg|s]
  w_Vehicle_CoG_dt[x;y;z][rad|s2] : BusSelector  OutputSignals=w_x_Vehicle_CoG_dt[rad|s2],w_y_Vehicle_CoG_dt[rad|s2],w_z_Vehicle_CoG_dt[rad|s2]
  z_Wheel_dt[FL;FR;RL;RR][m|s] : BusSelector  OutputSignals=z_FL_Wheel_dt[m|s],z_FR_Wheel_dt[m|s],z_RL_Wheel_dt[m|s],z_RR_Wheel_dt[m|s]
  wires:
  ASMSignalBus/1 -> BusSelector_1/1
  BusSelector_1/1 -> Control/1  "<Control>"
  Control/1 -> SoftECU_Brake/1  "<SoftECU_Brake>"
  SoftECU_Brake/1 -> DesiredBrakePressure/1  "<DesiredBrakePressure>"
  Control/2 -> SoftECU_PowerSteering/1  "<SoftECU_PowerSteering>"
  BusSelector_1/2 -> Plant/1  "<Plant>"
  Plant/1 -> VehicleMovement/1  "<VehicleMovement>"
  VehicleMovement/1 -> Accelerations/1  "<Accelerations>"
  Accelerations/1 -> VehicleCoG/1  "<VehicleCoG>"
  VehicleCoG/1 -> Linear/1  "<Linear>"
  Linear/1 -> a_Vehicle_CoG[x;y;z][m|s2]/1  "<a_Vehicle_CoG[x;y;z][m|s2]>"
  VehicleCoG/2 -> Angular/1  "<Angular>"
  Angular/1 -> w_Vehicle_CoG_dt[x;y;z][rad|s2]/1  "<w_Vehicle_CoG_dt[x;y;z][rad|s2]>"
  Accelerations/2 -> Wheels/1  "<Wheels>"
  Wheels/1 -> Linear1/1  "<Linear>"
  VehicleMovement/2 -> Velocities/1  "<Velocities>"
  Velocities/1 -> Vehicle/1  "<Vehicle>"
  Vehicle/1 -> Linear2/1  "<Linear>"
  Linear2/1 -> v_Vehicle_CoG[x;y;z][km|h]/1  "<v_Vehicle_CoG[x;y;z][km|h]>"
  Vehicle/2 -> Angular1/1  "<Angular>"
  Angular1/1 -> w_Vehicle_CoG[x;y;z][deg|s]/1  "<w_Vehicle_CoG[x;y;z][deg|s]>"
  Velocities/2 -> Wheels1/1  "<Wheels>"
  Wheels1/1 -> Linear3/1  "<Linear>"
  Linear3/1 -> WheelBodyVelocity/1  "<WheelBodyVelocity>"
  Wheels1/2 -> Angular2/1  "<Angular>"
  Angular2/1 -> WheelBodyAngularVelocity/1  "<WheelBodyAngularVelocity>"
  Angular2/2 -> WheelAngularVelocity/1  "<WheelAngularVelocity>"
  Velocities/3 -> Generalized/1  "<Generalized>"
  Generalized/3 -> z_Wheel_dt[FL;FR;RL;RR][m|s]/1  "<z_Wheel_dt[FL;FR;RL;RR][m|s]>"
  VehicleMovement/3 -> Positions/1  "<Positions>"
  Positions/1 -> Vehicle1/1  "<Vehicle>"
  Vehicle1/1 -> Linear4/1  "<Linear>"
  Linear4/1 -> Pos_Vehicle_CoorSys_E[x;y;z][m]/1  "<Pos_Vehicle_CoorSys_E[x;y;z][m]>"
  Vehicle1/2 -> Angular3/1  "<Angular>"
  Angular3/1 -> Angle_Vehicle_CoorSys_E[x;y;z][deg]/1  "<Angle_Vehicle_CoorSys_E[x;y;z][deg]>"
  Positions/2 -> Wheels2/1  "<Wheels>"
  Wheels2/1 -> Linear5/1  "<Linear>"
  VehicleMovement/4 -> VehicleEquationOfMotion/1  "<VehicleEquationOfMotion>"
  VehicleEquationOfMotion/1 -> GeneralizedForcesAndTorques/1  "<GeneralizedForcesAndTorques>"
  VehicleEquationOfMotion/2 -> GeneralizedVelocitiesDerivative/1  "<GeneralizedVelocitiesDerivative>"
  VehicleMovement/5 -> GravityAcceleration/1  "<GravityAcceleration>"
  VehicleMovement/6 -> SensorMotion/1  "<SensorMotion>"
  SensorMotion/1 -> Sensor1/1  "<Sensor1>"
  SensorMotion/2 -> Sensor2/1  "<Sensor2>"
  SensorMotion/3 -> Sensor3/1  "<Sensor3>"
  SensorMotion/4 -> Sensor4/1  "<Sensor4>"
  VehicleMovement/7 -> VehicleMassAndAdditionalLoads/1  "<VehicleMassAndAdditionalLoads>"
  VehicleMovement/8 -> MassForcesAndTorques/1  "<MassForcesAndTorques>"
  MassForcesAndTorques/1 -> GravitationalForces/1  "<GravitationalForces>"
  MassForcesAndTorques/2 -> GyroscopicForces/1  "<GyroscopicForces>"
  MassForcesAndTorques/3 -> GyroscopicTorques/1  "<GyroscopicTorques>"
  MassForcesAndTorques/4 -> ResidualAccelerations/1  "<ResidualAccelerations>"
  Plant/2 -> Tire/1  "<Tire>"
  Tire/1 -> Tire_allSignals/1  "<Tire_allSignals>"
  Tire_allSignals/1 -> Tire_FL/1  "<Tire_FL>"
  Tire_FL/1 -> ContactPoint/1  "<ContactPoint>"
  Tire_FL/2 -> TireForcesAndTorques/1  "<TireForcesAndTorques>"
  TireForcesAndTorques/1 -> F_Tire_CoorSys_V[x;y;z][N]/1  "<F_Tire_CoorSys_V[x;y;z][N]>"
  TireForcesAndTorques/2 -> Trq_Tire_CoorSys_V[x;y;z][Nm]/1  "<Trq_Tire_CoorSys_V[x;y;z][Nm]>"
  Tire_FL/3 -> Tire1/1  "<Tire>"
  Tire_allSignals/2 -> Tire_FR/1  "<Tire_FR>"
  Tire_FR/1 -> ContactPoint1/1  "<ContactPoint>"
  Tire_FR/2 -> TireForcesAndTorques1/1  "<TireForcesAndTorques>"
  TireForcesAndTorques1/1 -> F_Tire_CoorSys_V[x;y;z][N]1/1  "<F_Tire_CoorSys_V[x;y;z][N]>"
  TireForcesAndTorques1/2 -> Trq_Tire_CoorSys_V[x;y;z][Nm]1/1  "<Trq_Tire_CoorSys_V[x;y;z][Nm]>"
  Tire_FR/3 -> Tire2/1  "<Tire>"
  Tire_allSignals/3 -> Tire_RL/1  "<Tire_RL>"
  Tire_RL/1 -> ContactPoint2/1  "<ContactPoint>"
  Tire_RL/2 -> TireForcesAndTorques2/1  "<TireForcesAndTorques>"
  TireForcesAndTorques2/1 -> F_Tire_CoorSys_V[x;y;z][N]2/1  "<F_Tire_CoorSys_V[x;y;z][N]>"
  TireForcesAndTorques2/2 -> Trq_Tire_CoorSys_V[x;y;z][Nm]2/1  "<Trq_Tire_CoorSys_V[x;y;z][Nm]>"
  Tire_RL/3 -> Tire3/1  "<Tire>"
  Tire_allSignals/4 -> Tire_RR/1  "<Tire_RR>"
  Tire_RR/1 -> ContactPoint3/1  "<ContactPoint>"
  Tire_RR/2 -> TireForcesAndTorques3/1  "<TireForcesAndTorques>"
  TireForcesAndTorques3/1 -> F_Tire_CoorSys_V[x;y;z][N]3/1  "<F_Tire_CoorSys_V[x;y;z][N]>"
  TireForcesAndTorques3/2 -> Trq_Tire_CoorSys_V[x;y;z][Nm]3/1  "<Trq_Tire_CoorSys_V[x;y;z][Nm]>"
  Tire_RR/3 -> Tire4/1  "<Tire>"
  Plant/3 -> Aerodynamics/1  "<Aerodynamics>"
  Aerodynamics/1 -> Forces/1  "<Forces>"
  Aerodynamics/2 -> Torques/1  "<Torques>"
  Aerodynamics/3 -> Coefficients/1  "<Coefficients>"
  Plant/4 -> Wheel/1  "<Wheel>"
  Wheel/1 -> WheelSpeed_CoorSys_V/1  "<WheelSpeed_CoorSys_V>"
  Wheel/2 -> ShaftsTorques_CoorSys_V/1  "<ShaftsTorques_CoorSys_V>"
  Wheel/3 -> TireWheelTorques/1  "<TireWheelTorques>"
  Wheel/4 -> WheelSpeed/1  "<WheelSpeed>"
  Wheel/5 -> WheelSpeed2/1  "<WheelSpeed2>"
  Wheel/6 -> RotationAngle/1  "<RotationAngle>"
  Plant/5 -> Steering/1  "<Steering>"
  Steering/5 -> ForcesAndTorques/1  "<ForcesAndTorques>"
  Steering/6 -> GeneralizedForcesAndTorques1/1  "<GeneralizedForcesAndTorques>"
  Steering/14 -> StatesSteeringSystem/1  "<StatesSteeringSystem>"
  Steering/16 -> SteeringWheelTorque/1  "<SteeringWheelTorque>"
  Plant/6 -> Brake/1  "<Brake>"
  Brake/1 -> MasterBrakeCylinder/1  "<MasterBrakeCylinder>"
  MasterBrakeCylinder/2 -> ActiveBrakeCylinder/1  "<ActiveBrakeCylinder>"
  MasterBrakeCylinder/3 -> BrakeCylinderLinear/1  "<BrakeCylinderLinear>"
  MasterBrakeCylinder/4 -> BrakeCylinderPhysical/1  "<BrakeCylinderPhysical>"
  Brake/2 -> BrakeHydraulics/1  "<BrakeHydraulics>"
  BrakeHydraulics/1 -> BrakingCircuit/1  "<BrakingCircuit>"
  BrakingCircuit/1 -> Pressure/1  "<Pressure>"
  Brake/3 -> BrakeDisc/1  "<BrakeDisc>"
  BrakeDisc/1 -> Torque/1  "<Torque>"
  BrakeDisc/2 -> MaximumTorque/1  "<MaximumTorque>"
  BrakeDisc/3 -> Pressure1/1  "<Pressure>"
  BrakeDisc/4 -> Const_BrakeDiscFactor/1  "<Const_BrakeDiscFactor>"
  Brake/4 -> VacuumServo/1  "<VacuumServo>"
  VacuumServo/1 -> ManifoldValve/1  "<ManifoldValve>"
  VacuumServo/2 -> VacuumChamber/1  "<VacuumChamber>"
  VacuumServo/3 -> BellValve/1  "<BellValve>"
  VacuumServo/4 -> RearChamber/1  "<RearChamber>"
  VacuumServo/5 -> PushRod/1  "<PushRod>"
  PushRod/9 -> OutputPoint/1  "<OutputPoint>"
  VacuumServo/6 -> ControllerBellValve/1  "<ControllerBellValve>"
  Brake/5 -> Manifold/1  "<Manifold>"
  Plant/7 -> Suspension/1  "<Suspension>"
  Suspension/1 -> SuspensionFront/1  "<SuspensionFront>"
  SuspensionFront/1 -> SuspensionKinematicsFront/1  "<SuspensionKinematicsFront>"
  SuspensionKinematicsFront/1 -> Kinematics_Left/1  "<Kinematics_Left>"
  Kinematics_Left/1 -> Position_Left/1  "<Position_Left>"
  Kinematics_Left/2 -> Orientation_Left/1  "<Orientation_Left>"
  Orientation_Left/1 -> Angle_Left_Wheel[Alpha;Beta;Gamma][deg]/1  "<Angle_Left_Wheel[Alpha;Beta;Gamma][deg]>"
  Kinematics_Left/3 -> Spring_Left/1  "<Spring_Left>"
  Kinematics_Left/4 -> Damper_Left/1  "<Damper_Left>"
  SuspensionKinematicsFront/2 -> Kinematics_Right/1  "<Kinematics_Right>"
  Kinematics_Right/1 -> Position_Right/1  "<Position_Right>"
  Kinematics_Right/2 -> Orientation_Right/1  "<Orientation_Right>"
  Orientation_Right/1 -> Angle_Right_Wheel[Alpha;Beta;Gamma][deg]/1  "<Angle_Right_Wheel[Alpha;Beta;Gamma][deg]>"
  Kinematics_Right/3 -> Spring_Right/1  "<Spring_Right>"
  Kinematics_Right/4 -> Damper_Right/1  "<Damper_Right>"
  SuspensionKinematicsFront/3 -> Stabilizer/1  "<Stabilizer>"
  SuspensionFront/2 -> SuspensionComplianceFront/1  "<SuspensionComplianceFront>"
  SuspensionComplianceFront/9 -> ComplianceLongForce/1  "<ComplianceLongForce>"
  SuspensionComplianceFront/10 -> ComplianceLatForce/1  "<ComplianceLatForce>"
  SuspensionComplianceFront/11 -> ComplianceAligningTorque/1  "<ComplianceAligningTorque>"
  SuspensionComplianceFront/12 -> ComplianceLongTorque/1  "<ComplianceLongTorque>"
  SuspensionFront/3 -> SuspensionForcesFront/1  "<SuspensionForcesFront>"
  SuspensionFront/4 -> RelativePositionFront/1  "<RelativePositionFront>"
  RelativePositionFront/1 -> Pos_Wheel[FL;FR][x;y;z][m]/1  "<Pos_Wheel[FL;FR][x;y;z][m]>"
  RelativePositionFront/2 -> UnitVec_y_Wheel_CoorSys_V[FL;FR][x;y;z]/1  "<UnitVec_y_Wheel_CoorSys_V[FL;FR][x;y;z]>"
  RelativePositionFront/3 -> Angle_Wheel[FL;FR][Toe;Camber][deg]/1  "<Angle_Wheel[FL;FR][Toe;Camber][deg]>"
  Angle_Wheel[FL;FR][Toe;Camber][deg]/1 -> Angle_FL_Wheel[Toe;Camber][deg]/1  "<Angle_FL_Wheel[Toe;Camber][deg]>"
  Angle_Wheel[FL;FR][Toe;Camber][deg]/2 -> Angle_FR_Wheel[Toe;Camber][deg]/1  "<Angle_FR_Wheel[Toe;Camber][deg]>"
  Suspension/2 -> SuspensionRear/1  "<SuspensionRear>"
  SuspensionRear/1 -> SuspensionKinematicsRear/1  "<SuspensionKinematicsRear>"
  SuspensionKinematicsRear/1 -> Kinematics_Left1/1  "<Kinematics_Left>"
  Kinematics_Left1/1 -> Position_Left1/1  "<Position_Left>"
  Kinematics_Left1/2 -> Orientation_Left1/1  "<Orientation_Left>"
  Orientation_Left1/1 -> Angle_Left_Wheel[Alpha;Beta;Gamma][deg]1/1  "<Angle_Left_Wheel[Alpha;Beta;Gamma][deg]>"
  Kinematics_Left1/3 -> Spring_Left1/1  "<Spring_Left>"
  Kinematics_Left1/4 -> Damper_Left1/1  "<Damper_Left>"
  SuspensionKinematicsRear/2 -> Kinematics_Right1/1  "<Kinematics_Right>"
  Kinematics_Right1/1 -> Position_Right1/1  "<Position_Right>"
  Kinematics_Right1/2 -> Orientation_Right1/1  "<Orientation_Right>"
  Orientation_Right1/1 -> Angle_Right_Wheel[Alpha;Beta;Gamma][deg]1/1  "<Angle_Right_Wheel[Alpha;Beta;Gamma][deg]>"
  Kinematics_Right1/3 -> Spring_Right1/1  "<Spring_Right>"
  Kinematics_Right1/4 -> Damper_Right1/1  "<Damper_Right>"
  SuspensionKinematicsRear/3 -> Stabilizer1/1  "<Stabilizer>"
  SuspensionRear/2 -> SuspensionComplianceRear/1  "<SuspensionComplianceRear>"
  SuspensionComplianceRear/9 -> ComplianceLongForce1/1  "<ComplianceLongForce>"
  SuspensionComplianceRear/10 -> ComplianceLatForce1/1  "<ComplianceLatForce>"
  SuspensionComplianceRear/11 -> ComplianceAligningTorque1/1  "<ComplianceAligningTorque>"
  SuspensionComplianceRear/12 -> ComplianceLongTorque1/1  "<ComplianceLongTorque>"
  SuspensionRear/3 -> SuspensionForcesRear/1  "<SuspensionForcesRear>"
  SuspensionRear/4 -> RelativePositionRear/1  "<RelativePositionRear>"
  RelativePositionRear/1 -> Pos_Wheel[RL;RR][x;y;z][m]/1  "<Pos_Wheel[RL;RR][x;y;z][m]>"
  RelativePositionRear/2 -> UnitVec_y_Wheel_CoorSys_V[RL;RR][x;y;z]/1  "<UnitVec_y_Wheel_CoorSys_V[RL;RR][x;y;z]>"
  RelativePositionRear/3 -> Angle_Wheel[RL;RR][Toe;Camber][deg]/1  "<Angle_Wheel[RL;RR][Toe;Camber][deg]>"
  Angle_Wheel[RL;RR][Toe;Camber][deg]/1 -> Angle_RL_Wheel[Toe;Camber][deg]/1  "<Angle_RL_Wheel[Toe;Camber][deg]>"
  Angle_Wheel[RL;RR][Toe;Camber][deg]/2 -> Angle_RR_Wheel[Toe;Camber][deg]/1  "<Angle_RR_Wheel[Toe;Camber][deg]>"
  Plant/8 -> SteeringRod_Back_Calc/1  "<SteeringRod_Back_Calc>"
  Plant/9 -> DrivingResistances/1  "<DrivingResistances>"
  ContentID/1 -> Terminator/1
  DesiredBrakePressure/1 -> SignalFilter/1  "<Enable_p_Brake_Desired[0|1]>"
  DesiredBrakePressure/2 -> SignalFilter/2  "<p_Brake_Desired[bar]>"
  SoftECU_PowerSteering/1 -> SignalFilter/3  "<Trq_PowerSteering[Nm]>"
  a_Vehicle_CoG[x;y;z][m|s2]/1 -> SignalFilter/4  "<a_x_Vehicle_CoG[m|s2]>"
  a_Vehicle_CoG[x;y;z][m|s2]/2 -> SignalFilter/5  "<a_y_Vehicle_CoG[m|s2]>"
  a_Vehicle_CoG[x;y;z][m|s2]/3 -> SignalFilter/6  "<a_z_Vehicle_CoG[m|s2]>"
  Linear/2 -> Reshape_7/1  "<a_Vehicle_CoG_withG[x;y;z][m|s2]>"
  Reshape_7/1 -> SignalFilter/7
  w_Vehicle_CoG_dt[x;y;z][rad|s2]/1 -> SignalFilter/8  "<w_x_Vehicle_CoG_dt[rad|s2]>"
  w_Vehicle_CoG_dt[x;y;z][rad|s2]/2 -> SignalFilter/9  "<w_y_Vehicle_CoG_dt[rad|s2]>"
  w_Vehicle_CoG_dt[x;y;z][rad|s2]/3 -> SignalFilter/10  "<w_z_Vehicle_CoG_dt[rad|s2]>"
  Linear1/1 -> Reshape_11/1  "<a_FL_Wheel[x;y;z][m|s2]>"
  Reshape_11/1 -> SignalFilter/11
  Linear1/2 -> Reshape_12/1  "<a_FR_Wheel[x;y;z][m|s2]>"
  Reshape_12/1 -> SignalFilter/12
  Linear1/3 -> Reshape_13/1  "<a_RL_Wheel[x;y;z][m|s2]>"
  Reshape_13/1 -> SignalFilter/13
  Linear1/4 -> Reshape_14/1  "<a_RR_Wheel[x;y;z][m|s2]>"
  Reshape_14/1 -> SignalFilter/14
  v_Vehicle_CoG[x;y;z][km|h]/1 -> SignalFilter/15  "<v_x_Vehicle_CoG[km|h]>"
  v_Vehicle_CoG[x;y;z][km|h]/2 -> SignalFilter/16  "<v_y_Vehicle_CoG[km|h]>"
  v_Vehicle_CoG[x;y;z][km|h]/3 -> SignalFilter/17  "<v_z_Vehicle_CoG[km|h]>"
  Linear2/2 -> SignalFilter/18  "<v_Total_Vehicle[km|h]>"
  Linear2/3 -> SignalFilter/19  "<Angle_SideSlip_Vehicle[deg]>"
  w_Vehicle_CoG[x;y;z][deg|s]/1 -> SignalFilter/20  "<RollRate_Vehicle_CoG[deg|s]>"
  w_Vehicle_CoG[x;y;z][deg|s]/2 -> SignalFilter/21  "<PitchRate_Vehicle_CoG[deg|s]>"
  w_Vehicle_CoG[x;y;z][deg|s]/3 -> SignalFilter/22  "<YawRate_Vehicle_CoG[deg|s]>"
  WheelBodyVelocity/1 -> Reshape_23/1  "<v_FL_Abs_WheelBody[x;y;z][km|h]>"
  Reshape_23/1 -> SignalFilter/23
  WheelBodyVelocity/2 -> Reshape_24/1  "<v_FR_Abs_WheelBody[x;y;z][km|h]>"
  Reshape_24/1 -> SignalFilter/24
  WheelBodyVelocity/3 -> Reshape_25/1  "<v_RL_Abs_WheelBody[x;y;z][km|h]>"
  Reshape_25/1 -> SignalFilter/25
  WheelBodyVelocity/4 -> Reshape_26/1  "<v_RR_Abs_WheelBody[x;y;z][km|h]>"
  Reshape_26/1 -> SignalFilter/26
  WheelBodyAngularVelocity/1 -> Reshape_27/1  "<w_FL_Abs_WheelBody[x;y;z][rad|s]>"
  Reshape_27/1 -> SignalFilter/27
  WheelBodyAngularVelocity/2 -> Reshape_28/1  "<w_FR_Abs_WheelBody[x;y;z][rad|s]>"
  Reshape_28/1 -> SignalFilter/28
  WheelBodyAngularVelocity/3 -> Reshape_29/1  "<w_RL_Abs_WheelBody[x;y;z][rad|s]>"
  Reshape_29/1 -> SignalFilter/29
  WheelBodyAngularVelocity/4 -> Reshape_30/1  "<w_RR_Abs_WheelBody[x;y;z][rad|s]>"
  Reshape_30/1 -> SignalFilter/30
  WheelAngularVelocity/1 -> Reshape_31/1  "<w_FL_Abs_Wheel[x;y;z][rad|s]>"
  Reshape_31/1 -> SignalFilter/31
  WheelAngularVelocity/2 -> Reshape_32/1  "<w_FR_Abs_Wheel[x;y;z][rad|s]>"
  Reshape_32/1 -> SignalFilter/32
  WheelAngularVelocity/3 -> Reshape_33/1  "<w_RL_Abs_Wheel[x;y;z][rad|s]>"
  Reshape_33/1 -> SignalFilter/33
  WheelAngularVelocity/4 -> Reshape_34/1  "<w_RR_Abs_Wheel[x;y;z][rad|s]>"
  Reshape_34/1 -> SignalFilter/34
  Generalized/1 -> Reshape_35/1  "<v_Vehicle[x;y;z][km|h]>"
  Reshape_35/1 -> SignalFilter/35
  Generalized/2 -> Reshape_36/1  "<w_Vehicle[x;y;z][deg|s]>"
  Reshape_36/1 -> SignalFilter/36
  z_Wheel_dt[FL;FR;RL;RR][m|s]/1 -> SignalFilter/37  "<z_FL_Wheel_dt[m|s]>"
  z_Wheel_dt[FL;FR;RL;RR][m|s]/2 -> SignalFilter/38  "<z_FR_Wheel_dt[m|s]>"
  z_Wheel_dt[FL;FR;RL;RR][m|s]/3 -> SignalFilter/39  "<z_RL_Wheel_dt[m|s]>"
  z_Wheel_dt[FL;FR;RL;RR][m|s]/4 -> SignalFilter/40  "<z_RR_Wheel_dt[m|s]>"
  Pos_Vehicle_CoorSys_E[x;y;z][m]/1 -> SignalFilter/41  "<Pos_x_Vehicle_CoorSys_E[m]>"
  Pos_Vehicle_CoorSys_E[x;y;z][m]/2 -> SignalFilter/42  "<Pos_y_Vehicle_CoorSys_E[m]>"
  Pos_Vehicle_CoorSys_E[x;y;z][m]/3 -> SignalFilter/43  "<Pos_z_Vehicle_CoorSys_E[m]>"
  Linear4/2 -> Reshape_44/1  "<Pos_Vehicle_CoorSys_E[m]>"
  Reshape_44/1 -> SignalFilter/44
  Linear4/3 -> SignalFilter/45  "<s_Vehicle[m]>"
  Angle_Vehicle_CoorSys_E[x;y;z][deg]/1 -> SignalFilter/46  "<Angle_Roll_Vehicle_CoorSys_E[deg]>"
  Angle_Vehicle_CoorSys_E[x;y;z][deg]/2 -> SignalFilter/47  "<Angle_Pitch_Vehicle_CoorSys_E[deg]>"
  Angle_Vehicle_CoorSys_E[x;y;z][deg]/3 -> SignalFilter/48  "<Angle_Yaw_Vehicle_CoorSys_E[deg]>"
  Angular3/2 -> Reshape_49/1  "<Angle_V[Alpha;Beta;Gamma][deg]>"
  Reshape_49/1 -> SignalFilter/49
  Angular3/3 -> Reshape_50/1  "<RotationMatrix_V_to_E[3x3]>"
  Reshape_50/1 -> SignalFilter/50
  Angular3/4 -> Reshape_51/1  "<RotationMatrix_V_to_E[1x9]>"
  Reshape_51/1 -> SignalFilter/51
  Angular3/5 -> Reshape_52/1  "<RotationMatrix_V_to_E_T[3x3]>"
  Reshape_52/1 -> SignalFilter/52
  Angular3/6 -> Reshape_53/1  "<RotationMatrix_V_to_E_T[1x9]>"
  Reshape_53/1 -> SignalFilter/53
  Linear5/1 -> Reshape_54/1  "<Pos_FL_Wheels_CoorSys_E[x;y;z][m]>"
  Reshape_54/1 -> SignalFilter/54
  Linear5/2 -> Reshape_55/1  "<Pos_FR_Wheels_CoorSys_E[x;y;z][m]>"
  Reshape_55/1 -> SignalFilter/55
  Linear5/3 -> Reshape_56/1  "<Pos_RL_Wheels_CoorSys_E[x;y;z][m]>"
  Reshape_56/1 -> SignalFilter/56
  Linear5/4 -> Reshape_57/1  "<Pos_RR_Wheels_CoorSys_E[x;y;z][m]>"
  Reshape_57/1 -> SignalFilter/57
  GeneralizedForcesAndTorques/1 -> Reshape_58/1  "<g_F_Vehicle[x;y;z][N]>"
  Reshape_58/1 -> SignalFilter/58
  GeneralizedForcesAndTorques/2 -> Reshape_59/1  "<g_Trq_Vehicle[x;y;z][Nm]>"
  Reshape_59/1 -> SignalFilter/59
  GeneralizedForcesAndTorques/3 -> Reshape_60/1  "<g_F_z_Wheel[FL;FR;RL;RR][N]>"
  Reshape_60/1 -> SignalFilter/60
  GeneralizedVelocitiesDerivative/1 -> Reshape_61/1  "<v_Vehicle_dt[x;y;z][m|s2]>"
  Reshape_61/1 -> SignalFilter/61
  GeneralizedVelocitiesDerivative/2 -> Reshape_62/1  "<w_Vehicle_dt[x;y;z][rad|s2]>"
  Reshape_62/1 -> SignalFilter/62
  GeneralizedVelocitiesDerivative/3 -> Reshape_63/1  "<q_Wheel_dt2[q1_Front;q2_Front;q1_Rear;q2_Rear][]>"
  Reshape_63/1 -> SignalFilter/63
  GravityAcceleration/1 -> Reshape_64/1  "<a_Gravity_CoorSys_V[x;y;z][m|s2]>"
  Reshape_64/1 -> SignalFilter/64
  Sensor1/1 -> Reshape_65/1  "<a_Angular_Sensor1_CoorSys_V[x;y;z][rad|s2]>"
  Reshape_65/1 -> SignalFilter/65
  Sensor1/2 -> Reshape_66/1  "<a_Total_Sensor1_CoorSys_V[x;y;z][m|s2]>"
  Reshape_66/1 -> SignalFilter/66
  Sensor1/3 -> Reshape_67/1  "<a_Sensor1_CoorSys_V[x;y;z][m|s2]>"
  Reshape_67/1 -> SignalFilter/67
  Sensor1/4 -> Reshape_68/1  "<v_Sensor1_CoorSys_V[x;y;z][m|s]>"
  Reshape_68/1 -> SignalFilter/68
  Sensor1/5 -> Reshape_69/1  "<w_Sensor1_CoorSys_V[x;y;z][rad|s]>"
  Reshape_69/1 -> SignalFilter/69
  Sensor1/6 -> Reshape_70/1  "<a_Angular_Sensor1_CoorSys_VH[x;y;z][rad|s2]>"
  Reshape_70/1 -> SignalFilter/70
  Sensor1/7 -> Reshape_71/1  "<a_Total_Sensor1_CoorSys_VH[x;y;z][m|s2]>"
  Reshape_71/1 -> SignalFilter/71
  Sensor1/8 -> Reshape_72/1  "<a_Sensor1_CoorSys_VH[x;y;z][m|s2]>"
  Reshape_72/1 -> SignalFilter/72
  Sensor1/9 -> Reshape_73/1  "<v_Sensor1_CoorSys_VH[x;y;z][m|s]>"
  Reshape_73/1 -> SignalFilter/73
  Sensor1/10 -> Reshape_74/1  "<w_Sensor1_CoorSys_VH[x;y;z][rad|s]>"
  Reshape_74/1 -> SignalFilter/74
  Sensor2/1 -> Reshape_75/1  "<a_Angular_Sensor2_CoorSys_V[x;y;z][rad|s2]>"
  Reshape_75/1 -> SignalFilter/75
  Sensor2/2 -> Reshape_76/1  "<a_Total_Sensor2_CoorSys_V[x;y;z][m|s2]>"
  Reshape_76/1 -> SignalFilter/76
  Sensor2/3 -> Reshape_77/1  "<a_Sensor2_CoorSys_V[x;y;z][m|s2]>"
  Reshape_77/1 -> SignalFilter/77
  Sensor2/4 -> Reshape_78/1  "<v_Sensor2_CoorSys_V[x;y;z][m|s]>"
  Reshape_78/1 -> SignalFilter/78
  Sensor2/5 -> Reshape_79/1  "<w_Sensor2_CoorSys_V[x;y;z][rad|s]>"
  Reshape_79/1 -> SignalFilter/79
  Sensor2/6 -> Reshape_80/1  "<a_Angular_Sensor2_CoorSys_VH[x;y;z][rad|s2]>"
  Reshape_80/1 -> SignalFilter/80
  Sensor2/7 -> Reshape_81/1  "<a_Total_Sensor2_CoorSys_VH[x;y;z][m|s2]>"
  Reshape_81/1 -> SignalFilter/81
  Sensor2/8 -> Reshape_82/1  "<a_Sensor2_CoorSys_VH[x;y;z][m|s2]>"
  Reshape_82/1 -> SignalFilter/82
  Sensor2/9 -> Reshape_83/1  "<v_Sensor2_CoorSys_VH[x;y;z][m|s]>"
  Reshape_83/1 -> SignalFilter/83
  Sensor2/10 -> Reshape_84/1  "<w_Sensor2_CoorSys_VH[x;y;z][rad|s]>"
  Reshape_84/1 -> SignalFilter/84
  Sensor3/1 -> Reshape_85/1  "<a_Angular_Sensor3_CoorSys_V[x;y;z][rad|s2]>"
  Reshape_85/1 -> SignalFilter/85
  Sensor3/2 -> Reshape_86/1  "<a_Total_Sensor3_CoorSys_V[x;y;z][m|s2]>"
  Reshape_86/1 -> SignalFilter/86
  Sensor3/3 -> Reshape_87/1  "<a_Sensor3_CoorSys_V[x;y;z][m|s2]>"
  Reshape_87/1 -> SignalFilter/87
  Sensor3/4 -> Reshape_88/1  "<v_Sensor3_CoorSys_V[x;y;z][m|s]>"
  Reshape_88/1 -> SignalFilter/88
  Sensor3/5 -> Reshape_89/1  "<w_Sensor3_CoorSys_V[x;y;z][rad|s]>"
  Reshape_89/1 -> SignalFilter/89
  Sensor3/6 -> Reshape_90/1  "<a_Angular_Sensor3_CoorSys_VH[x;y;z][rad|s2]>"
  Reshape_90/1 -> SignalFilter/90
  Sensor3/7 -> Reshape_91/1  "<a_Total_Sensor3_CoorSys_VH[x;y;z][m|s2]>"
  Reshape_91/1 -> SignalFilter/91
  Sensor3/8 -> Reshape_92/1  "<a_Sensor3_CoorSys_VH[x;y;z][m|s2]>"
  Reshape_92/1 -> SignalFilter/92
  Sensor3/9 -> Reshape_93/1  "<v_Sensor3_CoorSys_VH[x;y;z][m|s]>"
  Reshape_93/1 -> SignalFilter/93
  Sensor3/10 -> Reshape_94/1  "<w_Sensor3_CoorSys_VH[x;y;z][rad|s]>"
  Reshape_94/1 -> SignalFilter/94
  Sensor4/1 -> Reshape_95/1  "<a_Angular_Sensor4_CoorSys_V[x;y;z][rad|s2]>"
  Reshape_95/1 -> SignalFilter/95
  Sensor4/2 -> Reshape_96/1  "<a_Total_Sensor4_CoorSys_V[x;y;z][m|s2]>"
  Reshape_96/1 -> SignalFilter/96
  Sensor4/3 -> Reshape_97/1  "<a_Sensor4_CoorSys_V[x;y;z][m|s2]>"
  Reshape_97/1 -> SignalFilter/97
  Sensor4/4 -> Reshape_98/1  "<v_Sensor4_CoorSys_V[x;y;z][m|s]>"
  Reshape_98/1 -> SignalFilter/98
  Sensor4/5 -> Reshape_99/1  "<w_Sensor4_CoorSys_V[x;y;z][rad|s]>"
  Reshape_99/1 -> SignalFilter/99
  Sensor4/6 -> Reshape_100/1  "<a_Angular_Sensor4_CoorSys_VH[x;y;z][rad|s2]>"
  Reshape_100/1 -> SignalFilter/100
  Sensor4/7 -> Reshape_101/1  "<a_Total_Sensor4_CoorSys_VH[x;y;z][m|s2]>"
  Reshape_101/1 -> SignalFilter/101
  Sensor4/8 -> Reshape_102/1  "<a_Sensor4_CoorSys_VH[x;y;z][m|s2]>"
  Reshape_102/1 -> SignalFilter/102
  Sensor4/9 -> Reshape_103/1  "<v_Sensor4_CoorSys_VH[x;y;z][m|s]>"
  Reshape_103/1 -> SignalFilter/103
  Sensor4/10 -> Reshape_104/1  "<w_Sensor4_CoorSys_VH[x;y;z][rad|s]>"
  Reshape_104/1 -> SignalFilter/104
  VehicleMassAndAdditionalLoads/1 -> SignalFilter/105  "<m_TotalVehicle[kg]>"
  VehicleMassAndAdditionalLoads/2 -> Reshape_106/1  "<PosVec_CoG_TotalVehicle[x;y;z][m]>"
  Reshape_106/1 -> SignalFilter/106
  VehicleMassAndAdditionalLoads/3 -> SignalFilter/107  "<Pos_x_CoG_Vehicle_Total[m]>"
  VehicleMassAndAdditionalLoads/4 -> Reshape_108/1  "<Inertia_Tensor_TotalVehicle[3x3][kgm2]>"
  Reshape_108/1 -> SignalFilter/108
  VehicleMassAndAdditionalLoads/5 -> SignalFilter/109  "<Inertia_z_Vehicle_Total[kgm2]>"
  VehicleMassAndAdditionalLoads/6 -> SignalFilter/110  "<m_TotalV1[kg]>"
  VehicleMassAndAdditionalLoads/7 -> Reshape_111/1  "<PosVec_CoG_TotalV1[x;y;z][m]>"
  Reshape_111/1 -> SignalFilter/111
  VehicleMassAndAdditionalLoads/8 -> Reshape_112/1  "<Inertia_Tensor_TotalV1[3x3][kgm2]>"
  Reshape_112/1 -> SignalFilter/112
  GravitationalForces/1 -> Reshape_113/1  "<F_Vehicle_Gravitational[x;y;z][N]>"
  Reshape_113/1 -> SignalFilter/113
  GravitationalForces/2 -> Reshape_114/1  "<F_FL_Gravitational[x;y;z][N]>"
  Reshape_114/1 -> SignalFilter/114
  GravitationalForces/3 -> Reshape_115/1  "<F_FR_Gravitational[x;y;z][N]>"
  Reshape_115/1 -> SignalFilter/115
  GravitationalForces/4 -> Reshape_116/1  "<F_RL_Gravitational[x;y;z][N]>"
  Reshape_116/1 -> SignalFilter/116
  GravitationalForces/5 -> Reshape_117/1  "<F_RR_Gravitational[x;y;z][N]>"
  Reshape_117/1 -> SignalFilter/117
  GyroscopicForces/1 -> Reshape_118/1  "<F_Vehicle_Gyroscopic[x;y;z][N]>"
  Reshape_118/1 -> SignalFilter/118
  GyroscopicForces/2 -> Reshape_119/1  "<F_FL_Gyroscopic[x;y;z][N]>"
  Reshape_119/1 -> SignalFilter/119
  GyroscopicForces/3 -> Reshape_120/1  "<F_FR_Gyroscopic[x;y;z][N]>"
  Reshape_120/1 -> SignalFilter/120
  GyroscopicForces/4 -> Reshape_121/1  "<F_RL_Gyroscopic[x;y;z][N]>"
  Reshape_121/1 -> SignalFilter/121
  GyroscopicForces/5 -> Reshape_122/1  "<F_RR_Gyroscopic[x;y;z][N]>"
  Reshape_122/1 -> SignalFilter/122
  GyroscopicTorques/1 -> Reshape_123/1  "<Trq_Vehicle_Gyroscope[x;y;z][Nm]>"
  Reshape_123/1 -> SignalFilter/123
  GyroscopicTorques/2 -> Reshape_124/1  "<Trq_FL_Gyroscope[x;y;z][Nm]>"
  Reshape_124/1 -> SignalFilter/124
  GyroscopicTorques/3 -> Reshape_125/1  "<Trq_FR_Gyroscope[x;y;z][Nm]>"
  Reshape_125/1 -> SignalFilter/125
  GyroscopicTorques/4 -> Reshape_126/1  "<Trq_RL_Gyroscope[x;y;z][Nm]>"
  Reshape_126/1 -> SignalFilter/126
  GyroscopicTorques/5 -> Reshape_127/1  "<Trq_RR_Gyroscope[x;y;z][Nm]>"
  Reshape_127/1 -> SignalFilter/127
  ResidualAccelerations/1 -> Reshape_128/1  "<a_Vehicle_CoG_Residual[x;y;z][m|s2]>"
  Reshape_128/1 -> SignalFilter/128
  ResidualAccelerations/2 -> Reshape_129/1  "<a_FL_Residual[x;y;z][m|s2]>"
  Reshape_129/1 -> SignalFilter/129
  ResidualAccelerations/3 -> Reshape_130/1  "<a_FR_Residual[x;y;z][m|s2]>"
  Reshape_130/1 -> SignalFilter/130
  ResidualAccelerations/4 -> Reshape_131/1  "<a_RL_Residual[x;y;z][m|s2]>"
  Reshape_131/1 -> SignalFilter/131
  ResidualAccelerations/5 -> Reshape_132/1  "<a_RR_Residual[x;y;z][m|s2]>"
  Reshape_132/1 -> SignalFilter/132
  ContactPoint/1 -> SignalFilter/133  "<r_Tire[m]>"
  ContactPoint/2 -> Reshape_134/1  "<Pos_CP_CoorSys_E[x;y][m]>"
  Reshape_134/1 -> SignalFilter/134
  F_Tire_CoorSys_V[x;y;z][N]/1 -> SignalFilter/135  "<F_x_Tire_CoorSys_V[N]>"
  F_Tire_CoorSys_V[x;y;z][N]/2 -> SignalFilter/136  "<F_y_Tire_CoorSys_V[N]>"
  F_Tire_CoorSys_V[x;y;z][N]/3 -> SignalFilter/137  "<F_z_Tire_CoorSys_V[N]>"
  Trq_Tire_CoorSys_V[x;y;z][Nm]/1 -> SignalFilter/138  "<Trq_x_Tire_CoorSys_V[Nm]>"
  Trq_Tire_CoorSys_V[x;y;z][Nm]/2 -> SignalFilter/139  "<Trq_y_Tire_CoorSys_V[Nm]>"
  Trq_Tire_CoorSys_V[x;y;z][Nm]/3 -> SignalFilter/140  "<Trq_z_Tire_CoorSys_V[Nm]>"
  Tire1/1 -> SignalFilter/141  "<v_Circumf_Dyn_Wheel[km|h]>"
  Tire1/2 -> SignalFilter/142  "<Slip_x[]>"
  Tire1/3 -> SignalFilter/143  "<Slip_y[]>"
  Tire1/4 -> SignalFilter/144  "<r_Dyn_Tire[m]>"
  Tire1/5 -> SignalFilter/145  "<CorneringStiffness[N|rad]>"
  Tire1/6 -> SignalFilter/146  "<Coef_RollingRes[]>"
  Tire1/7 -> SignalFilter/147  "<Trq_x_CoorSys_CP[Nm]>"
  Tire1/8 -> SignalFilter/148  "<Trq_y_CoorSys_W[Nm]>"
  Tire1/9 -> SignalFilter/149  "<Trq_z_CoorSys_CP[Nm]>"
  Tire1/10 -> SignalFilter/150  "<F_x_Dyn_Tire_CoorSys_CP[N]>"
  Tire1/11 -> SignalFilter/151  "<F_y_Dyn_Tire_CoorSys_CP[N]>"
  Tire1/12 -> SignalFilter/152  "<F_z_Dyn_Tire_CoorSys_CP[N]>"
  Tire1/13 -> SignalFilter/153  "<Const_r_unloaded_Tire[m]>"
  Tire1/14 -> SignalFilter/154  "<Const_Stiffness_z_Tire[N|m]>"
  ContactPoint1/1 -> SignalFilter/155  "<r_Tire[m]>"
  ContactPoint1/2 -> Reshape_156/1  "<Pos_CP_CoorSys_E[x;y][m]>"
  Reshape_156/1 -> SignalFilter/156
  F_Tire_CoorSys_V[x;y;z][N]1/1 -> SignalFilter/157  "<F_x_Tire_CoorSys_V[N]>"
  F_Tire_CoorSys_V[x;y;z][N]1/2 -> SignalFilter/158  "<F_y_Tire_CoorSys_V[N]>"
  F_Tire_CoorSys_V[x;y;z][N]1/3 -> SignalFilter/159  "<F_z_Tire_CoorSys_V[N]>"
  Trq_Tire_CoorSys_V[x;y;z][Nm]1/1 -> SignalFilter/160  "<Trq_x_Tire_CoorSys_V[Nm]>"
  Trq_Tire_CoorSys_V[x;y;z][Nm]1/2 -> SignalFilter/161  "<Trq_y_Tire_CoorSys_V[Nm]>"
  Trq_Tire_CoorSys_V[x;y;z][Nm]1/3 -> SignalFilter/162  "<Trq_z_Tire_CoorSys_V[Nm]>"
  Tire2/1 -> SignalFilter/163  "<v_Circumf_Dyn_Wheel[km|h]>"
  Tire2/2 -> SignalFilter/164  "<Slip_x[]>"
  Tire2/3 -> SignalFilter/165  "<Slip_y[]>"
  Tire2/4 -> SignalFilter/166  "<r_Dyn_Tire[m]>"
  Tire2/5 -> SignalFilter/167  "<CorneringStiffness[N|rad]>"
  Tire2/6 -> SignalFilter/168  "<Coef_RollingRes[]>"
  Tire2/7 -> SignalFilter/169  "<Trq_x_CoorSys_CP[Nm]>"
  Tire2/8 -> SignalFilter/170  "<Trq_y_CoorSys_W[Nm]>"
  Tire2/9 -> SignalFilter/171  "<Trq_z_CoorSys_CP[Nm]>"
  Tire2/10 -> SignalFilter/172  "<F_x_Dyn_Tire_CoorSys_CP[N]>"
  Tire2/11 -> SignalFilter/173  "<F_y_Dyn_Tire_CoorSys_CP[N]>"
  Tire2/12 -> SignalFilter/174  "<F_z_Dyn_Tire_CoorSys_CP[N]>"
  Tire2/13 -> SignalFilter/175  "<Const_r_unloaded_Tire[m]>"
  Tire2/14 -> SignalFilter/176  "<Const_Stiffness_z_Tire[N|m]>"
  ContactPoint2/1 -> SignalFilter/177  "<r_Tire[m]>"
  ContactPoint2/2 -> Reshape_178/1  "<Pos_CP_CoorSys_E[x;y][m]>"
  Reshape_178/1 -> SignalFilter/178
  F_Tire_CoorSys_V[x;y;z][N]2/1 -> SignalFilter/179  "<F_x_Tire_CoorSys_V[N]>"
  F_Tire_CoorSys_V[x;y;z][N]2/2 -> SignalFilter/180  "<F_y_Tire_CoorSys_V[N]>"
  F_Tire_CoorSys_V[x;y;z][N]2/3 -> SignalFilter/181  "<F_z_Tire_CoorSys_V[N]>"
  Trq_Tire_CoorSys_V[x;y;z][Nm]2/1 -> SignalFilter/182  "<Trq_x_Tire_CoorSys_V[Nm]>"
  Trq_Tire_CoorSys_V[x;y;z][Nm]2/2 -> SignalFilter/183  "<Trq_y_Tire_CoorSys_V[Nm]>"
  Trq_Tire_CoorSys_V[x;y;z][Nm]2/3 -> SignalFilter/184  "<Trq_z_Tire_CoorSys_V[Nm]>"
  Tire3/1 -> SignalFilter/185  "<v_Circumf_Dyn_Wheel[km|h]>"
  Tire3/2 -> SignalFilter/186  "<Slip_x[]>"
  Tire3/3 -> SignalFilter/187  "<Slip_y[]>"
  Tire3/4 -> SignalFilter/188  "<r_Dyn_Tire[m]>"
  Tire3/5 -> SignalFilter/189  "<CorneringStiffness[N|rad]>"
  Tire3/6 -> SignalFilter/190  "<Coef_RollingRes[]>"
  Tire3/7 -> SignalFilter/191  "<Trq_x_CoorSys_CP[Nm]>"
  Tire3/8 -> SignalFilter/192  "<Trq_y_CoorSys_W[Nm]>"
  Tire3/9 -> SignalFilter/193  "<Trq_z_CoorSys_CP[Nm]>"
  Tire3/10 -> SignalFilter/194  "<F_x_Dyn_Tire_CoorSys_CP[N]>"
  Tire3/11 -> SignalFilter/195  "<F_y_Dyn_Tire_CoorSys_CP[N]>"
  Tire3/12 -> SignalFilter/196  "<F_z_Dyn_Tire_CoorSys_CP[N]>"
  Tire3/13 -> SignalFilter/197  "<Const_r_unloaded_Tire[m]>"
  Tire3/14 -> SignalFilter/198  "<Const_Stiffness_z_Tire[N|m]>"
  ContactPoint3/1 -> SignalFilter/199  "<r_Tire[m]>"
  ContactPoint3/2 -> Reshape_200/1  "<Pos_CP_CoorSys_E[x;y][m]>"
  Reshape_200/1 -> SignalFilter/200
  F_Tire_CoorSys_V[x;y;z][N]3/1 -> SignalFilter/201  "<F_x_Tire_CoorSys_V[N]>"
  F_Tire_CoorSys_V[x;y;z][N]3/2 -> SignalFilter/202  "<F_y_Tire_CoorSys_V[N]>"
  F_Tire_CoorSys_V[x;y;z][N]3/3 -> SignalFilter/203  "<F_z_Tire_CoorSys_V[N]>"
  Trq_Tire_CoorSys_V[x;y;z][Nm]3/1 -> SignalFilter/204  "<Trq_x_Tire_CoorSys_V[Nm]>"
  Trq_Tire_CoorSys_V[x;y;z][Nm]3/2 -> SignalFilter/205  "<Trq_y_Tire_CoorSys_V[Nm]>"
  Trq_Tire_CoorSys_V[x;y;z][Nm]3/3 -> SignalFilter/206  "<Trq_z_Tire_CoorSys_V[Nm]>"
  Tire4/1 -> SignalFilter/207  "<v_Circumf_Dyn_Wheel[km|h]>"
  Tire4/2 -> SignalFilter/208  "<Slip_x[]>"
  Tire4/3 -> SignalFilter/209  "<Slip_y[]>"
  Tire4/4 -> SignalFilter/210  "<r_Dyn_Tire[m]>"
  Tire4/5 -> SignalFilter/211  "<CorneringStiffness[N|rad]>"
  Tire4/6 -> SignalFilter/212  "<Coef_RollingRes[]>"
  Tire4/7 -> SignalFilter/213  "<Trq_x_CoorSys_CP[Nm]>"
  Tire4/8 -> SignalFilter/214  "<Trq_y_CoorSys_W[Nm]>"
  Tire4/9 -> SignalFilter/215  "<Trq_z_CoorSys_CP[Nm]>"
  Tire4/10 -> SignalFilter/216  "<F_x_Dyn_Tire_CoorSys_CP[N]>"
  Tire4/11 -> SignalFilter/217  "<F_y_Dyn_Tire_CoorSys_CP[N]>"
  Tire4/12 -> SignalFilter/218  "<F_z_Dyn_Tire_CoorSys_CP[N]>"
  Tire4/13 -> SignalFilter/219  "<Const_r_unloaded_Tire[m]>"
  Tire4/14 -> SignalFilter/220  "<Const_Stiffness_z_Tire[N|m]>"
  Tire/2 -> Reshape_221/1  "<r_Dyn_Tire[FL;FR;RL;RR][m]>"
  Reshape_221/1 -> SignalFilter/221
  Tire/3 -> SignalFilter/222  "<r_Dyn_Tire_Mean[m]>"
  Tire/4 -> Reshape_223/1  "<Coef_RollingRes[FL;FR;RL;RR][]>"
  Reshape_223/1 -> SignalFilter/223
  Tire/5 -> SignalFilter/224  "<Coef_RollingRes_Mean[]>"
  Tire/6 -> SignalFilter/225  "<CorneringStiffness_Tire_Front[N|rad]>"
  Tire/7 -> SignalFilter/226  "<CorneringStiffness_Tire_Rear[N|rad]>"
  Tire/8 -> Reshape_227/1  "<CorneringStiffness[FL;FR;RL;RR][N|rad]>"
  Reshape_227/1 -> SignalFilter/227
  Tire/9 -> Reshape_228/1  "<Const_r_unloaded_Tire[FL;FR;RL;RR][m]>"
  Reshape_228/1 -> SignalFilter/228
  Tire/10 -> SignalFilter/229  "<Const_r_unloaded_Tire_Mean[m]>"
  Tire/11 -> Reshape_230/1  "<Slip_x_Wheel[]>"
  Reshape_230/1 -> SignalFilter/230
  Forces/1 -> SignalFilter/231  "<F_x_Aero_CoorSys_V[N]>"
  Forces/2 -> SignalFilter/232  "<F_y_Aero_CoorSys_V[N]>"
  Forces/3 -> SignalFilter/233  "<F_z_Aero_CoorSys_V[N]>"
  Torques/1 -> SignalFilter/234  "<Trq_x_Aero_CoorSys_V[Nm]>"
  Torques/2 -> SignalFilter/235  "<Trq_y_Aero_CoorSys_V[Nm]>"
  Torques/3 -> SignalFilter/236  "<Trq_z_Aero_CoorSys_V[Nm]>"
  Coefficients/1 -> SignalFilter/237  "<Cw_x[]>"
  WheelSpeed_CoorSys_V/1 -> Reshape_238/1  "<w_Wheel_FL_CoorSys_V[x;y;z][rad|s]>"
  Reshape_238/1 -> SignalFilter/238
  WheelSpeed_CoorSys_V/2 -> Reshape_239/1  "<w_Wheel_FR_CoorSys_V[x;y;z][rad|s]>"
  Reshape_239/1 -> SignalFilter/239
  WheelSpeed_CoorSys_V/3 -> Reshape_240/1  "<w_Wheel_RL_CoorSys_V[x;y;z][rad|s]>"
  Reshape_240/1 -> SignalFilter/240
  WheelSpeed_CoorSys_V/4 -> Reshape_241/1  "<w_Wheel_RR_CoorSys_V[x;y;z][rad|s]>"
  Reshape_241/1 -> SignalFilter/241
  ShaftsTorques_CoorSys_V/1 -> Reshape_242/1  "<Trq_Shaft_FL_CoorSys_V[x;y;z][Nm]>"
  Reshape_242/1 -> SignalFilter/242
  ShaftsTorques_CoorSys_V/2 -> Reshape_243/1  "<Trq_Shaft_FR_CoorSys_V[x;y;z][Nm]>"
  Reshape_243/1 -> SignalFilter/243
  ShaftsTorques_CoorSys_V/3 -> Reshape_244/1  "<Trq_Shaft_RL_CoorSys_V[x;y;z][Nm]>"
  Reshape_244/1 -> SignalFilter/244
  ShaftsTorques_CoorSys_V/4 -> Reshape_245/1  "<Trq_Shaft_RR_CoorSys_V[x;y;z][Nm]>"
  Reshape_245/1 -> SignalFilter/245
  TireWheelTorques/1 -> SignalFilter/246  "<Trq_Tire_Wheel_FL[Nm]>"
  TireWheelTorques/2 -> SignalFilter/247  "<Trq_Tire_Wheel_FR[Nm]>"
  TireWheelTorques/3 -> SignalFilter/248  "<Trq_Tire_Wheel_RL[Nm]>"
  TireWheelTorques/4 -> SignalFilter/249  "<Trq_Tire_Wheel_RR[Nm]>"
  WheelSpeed/1 -> SignalFilter/250  "<omega_FL_Wheel[rad|s]>"
  WheelSpeed/2 -> SignalFilter/251  "<omega_FR_Wheel[rad|s]>"
  WheelSpeed/3 -> SignalFilter/252  "<omega_RL_Wheel[rad|s]>"
  WheelSpeed/4 -> SignalFilter/253  "<omega_RR_Wheel[rad|s]>"
  WheelSpeed2/1 -> Reshape_254/1  "<omega_Wheel[FL;FR;RL;RR][rad|s]>"
  Reshape_254/1 -> SignalFilter/254
  WheelSpeed2/2 -> SignalFilter/255  "<omega_Mean_Wheel[rad|s]>"
  RotationAngle/1 -> SignalFilter/256  "<Angle_Rot_FL_Wheel[deg]>"
  RotationAngle/2 -> SignalFilter/257  "<Angle_Rot_FR_Wheel[deg]>"
  RotationAngle/3 -> SignalFilter/258  "<Angle_Rot_RL_Wheel[deg]>"
  RotationAngle/4 -> SignalFilter/259  "<Angle_Rot_RR_Wheel[deg]>"
  Steering/1 -> SignalFilter/260  "<Displ_Steering[m]>"
  Steering/2 -> SignalFilter/261  "<Displ_Steering_dt[m|s]>"
  Steering/3 -> SignalFilter/262  "<Displ_SteeringRod_dt2[m|s2]>"
  Steering/4 -> SignalFilter/263  "<m_Steering[kg]>"
  ForcesAndTorques/1 -> SignalFilter/264  "<g_F_Steering_SteeringRod[N]>"
  ForcesAndTorques/2 -> SignalFilter/265  "<Trq_Steering[Nm]>"
  ForcesAndTorques/3 -> SignalFilter/266  "<Trq_PowerSteering[Nm]>"
  ForcesAndTorques/4 -> SignalFilter/267  "<TrqSpring_SteeringColumn[Nm]>"
  ForcesAndTorques/5 -> SignalFilter/268  "<Trq_PowerSteeringDynamics[Nm]>"
  ForcesAndTorques/6 -> SignalFilter/269  "<TrqSpring_PowerSteeringSystem[Nm]>"
  GeneralizedForcesAndTorques1/1 -> SignalFilter/270  "<g_FTrq_Tire_Steering[N]>"
  GeneralizedForcesAndTorques1/2 -> SignalFilter/271  "<g_Trq_FL_Steering[N]>"
  GeneralizedForcesAndTorques1/3 -> SignalFilter/272  "<g_Trq_FR_Steering[N]>"
  GeneralizedForcesAndTorques1/4 -> SignalFilter/273  "<g_F_FL_Steering[N]>"
  GeneralizedForcesAndTorques1/5 -> SignalFilter/274  "<g_F_FR_Steering[N]>"
  Steering/7 -> SignalFilter/275  "<i_Steering[rad|m]>"
  Steering/8 -> SignalFilter/276  "<i_Steering_Mean[]>"
  Steering/9 -> SignalFilter/277  "<Angle_SteeringGear[deg]>"
  Steering/10 -> SignalFilter/278  "<Angle_SteeringWheel[deg]>"
  Steering/11 -> SignalFilter/279  "<Angle_SteeringGear_dt[deg|s]>"
  Steering/12 -> SignalFilter/280  "<Angle_SteeringWheel_dt[deg|s]>"
  Steering/13 -> SignalFilter/281  "<Const_Stiffness_SteeringColumn[Nm|rad]>"
  StatesSteeringSystem/1 -> SignalFilter/282  "<Angle_EPSSystem[deg]>"
  StatesSteeringSystem/2 -> SignalFilter/283  "<Angle_EPSSystem_dt[deg|s]>"
  StatesSteeringSystem/3 -> SignalFilter/284  "<Angle_LowerSteeringColumn[deg]>"
  StatesSteeringSystem/4 -> SignalFilter/285  "<Angle_LowerSteeringColumn_dt[deg|s]>"
  StatesSteeringSystem/5 -> SignalFilter/286  "<Angle_UpperSteeringColumn[deg]>"
  StatesSteeringSystem/6 -> SignalFilter/287  "<Angle_UpperSteeringColumn_dt[deg|s]>"
  StatesSteeringSystem/7 -> SignalFilter/288  "<Angle_SteeringWheel[deg]>"
  StatesSteeringSystem/8 -> SignalFilter/289  "<Angle_SteeringWheel_dt[deg|s]>"
  StatesSteeringSystem/9 -> SignalFilter/290  "<Displ_Steering[m]>"
  StatesSteeringSystem/10 -> SignalFilter/291  "<Displ_Steering_dt[m|s]>"
  StatesSteeringSystem/11 -> SignalFilter/292  "<Displ_SteeringRod_dt2[m|s2]>"
  StatesSteeringSystem/12 -> SignalFilter/293  "<Angle_SteeringGear[deg]>"
  StatesSteeringSystem/13 -> SignalFilter/294  "<Angle_SteeringGear_dt[deg|s]>"
  StatesSteeringSystem/14 -> SignalFilter/295  "<Angle_EPSPinion[rad]>"
  StatesSteeringSystem/15 -> SignalFilter/296  "<Angle_EPSPinion_dt[rad|s]>"
  StatesSteeringSystem/16 -> SignalFilter/297  "<i_Steering[rad|m]>"
  StatesSteeringSystem/17 -> SignalFilter/298  "<FrictionForce_SteeringRod[N]>"
  StatesSteeringSystem/18 -> SignalFilter/299  "<i_Steering_Wheel2Rod[rad|m]>"
  Steering/15 -> SignalFilter/300  "<FrictionTrq_SteeringSystem[Nm]>"
  SteeringWheelTorque/1 -> SignalFilter/301  "<TrqSensor_Steering[Nm]>"
  SteeringWheelTorque/2 -> SignalFilter/302  "<Trq_Driver[Nm]>"
  SteeringWheelTorque/3 -> SignalFilter/303  "<g_Trq_SteeringWheel[Nm]>"
  SteeringWheelTorque/4 -> SignalFilter/304  "<TrqFriction_SteeringWheel[Nm]>"
  SteeringWheelTorque/5 -> SignalFilter/305  "<Trq_SteeringWheel[Nm]>"
  MasterBrakeCylinder/1 -> SignalFilter/306  "<Sw_MasterBrakeCylinder_Mode[1linear|2physical|3Booster|4BrakeByWire]>"
  ActiveBrakeCylinder/1 -> SignalFilter/307  "<p[bar]>"
  ActiveBrakeCylinder/2 -> SignalFilter/308  "<p_max[bar]>"
  ActiveBrakeCylinder/3 -> SignalFilter/309  "<Enable_p_Brake_Desired[0|1]>"
  ActiveBrakeCylinder/4 -> SignalFilter/310  "<p_Brake_Desired[bar]>"
  BrakeCylinderLinear/1 -> SignalFilter/311  "<p[bar]>"
  BrakeCylinderLinear/2 -> SignalFilter/312  "<p_max[bar]>"
  BrakeCylinderPhysical/1 -> SignalFilter/313  "<Displ_Piston[mm]>"
  BrakeCylinderPhysical/2 -> SignalFilter/314  "<F[N]>"
  BrakeCylinderPhysical/3 -> SignalFilter/315  "<p[bar]>"
  BrakeCylinderPhysical/4 -> SignalFilter/316  "<p_max[bar]>"
  Pressure/1 -> SignalFilter/317  "<p_FL_Brake[bar]>"
  Pressure/2 -> SignalFilter/318  "<p_FR_Brake[bar]>"
  Pressure/3 -> SignalFilter/319  "<p_RL_Brake[bar]>"
  Pressure/4 -> SignalFilter/320  "<p_RR_Brake[bar]>"
  BrakeHydraulics/2 -> SignalFilter/321  "<BrakeHydraulicsModel[]>"
  Torque/1 -> SignalFilter/322  "<Trq_FL_Brake[Nm]>"
  Torque/2 -> SignalFilter/323  "<Trq_FR_Brake[Nm]>"
  Torque/3 -> SignalFilter/324  "<Trq_RL_Brake[Nm]>"
  Torque/4 -> SignalFilter/325  "<Trq_RR_Brake[Nm]>"
  MaximumTorque/1 -> SignalFilter/326  "<Trq_Max_Brake[Nm]>"
  MaximumTorque/2 -> Reshape_327/1  "<Trq_Max_Brake[FL;FR;RL;RR][Nm]>"
  Reshape_327/1 -> SignalFilter/327
  MaximumTorque/3 -> SignalFilter/328  "<Trq_FL_max_Brake[Nm]>"
  MaximumTorque/4 -> SignalFilter/329  "<Trq_FR_max_Brake[Nm]>"
  MaximumTorque/5 -> SignalFilter/330  "<Trq_RL_max_Brake[Nm]>"
  MaximumTorque/6 -> SignalFilter/331  "<Trq_RR_max_Brake[Nm]>"
  Pressure1/1 -> SignalFilter/332  "<p_FL_Brake[bar]>"
  Pressure1/2 -> SignalFilter/333  "<p_FR_Brake[bar]>"
  Pressure1/3 -> SignalFilter/334  "<p_RL_Brake[bar]>"
  Pressure1/4 -> SignalFilter/335  "<p_RR_Brake[bar]>"
  Const_BrakeDiscFactor/1 -> SignalFilter/336  "<Const_BrakeDiscFactor_FL[m3]>"
  Const_BrakeDiscFactor/2 -> SignalFilter/337  "<Const_BrakeDiscFactor_FR[m3]>"
  Const_BrakeDiscFactor/3 -> SignalFilter/338  "<Const_BrakeDiscFactor_RL[m3]>"
  Const_BrakeDiscFactor/4 -> SignalFilter/339  "<Const_BrakeDiscFactor_RR[m3]>"
  ManifoldValve/1 -> SignalFilter/340  "<p_In_MainfoldValve[bar]>"
  ManifoldValve/2 -> SignalFilter/341  "<p_Out_MainfoldValve[bar]>"
  ManifoldValve/3 -> SignalFilter/342  "<T_In_MainfoldValve[degC]>"
  ManifoldValve/4 -> SignalFilter/343  "<m_dot_ManifoldValve[kg|s]>"
  ManifoldValve/5 -> SignalFilter/344  "<m_dot_Out_ManifoldValve[kg|s]>"
  ManifoldValve/6 -> SignalFilter/345  "<m_dot_In_ManifoldValve[kg|s]>"
  VacuumChamber/1 -> SignalFilter/346  "<m_dot_In_1_VacuumChamber[kg|s]>"
  VacuumChamber/2 -> SignalFilter/347  "<m_dot_In_2_VacuumChamber[kg|s]>"
  VacuumChamber/3 -> SignalFilter/348  "<m_dot_Out_2_VacuumChamber[kg|s]>"
  VacuumChamber/4 -> SignalFilter/349  "<T_VacuumChamber[degC]>"
  VacuumChamber/5 -> SignalFilter/350  "<p_VacuumChamber[bar]>"
  VacuumChamber/6 -> SignalFilter/351  "<V_VacuumChamber[m3]>"
  BellValve/1 -> SignalFilter/352  "<ValveState[1ChamberCon|2AmbientCon|3CloseAll]>"
  BellValve/2 -> SignalFilter/353  "<p_In_BellValve[bar]>"
  BellValve/3 -> SignalFilter/354  "<p_Out_BellValve[bar]>"
  BellValve/4 -> SignalFilter/355  "<T_In_BellValve[degC]>"
  BellValve/5 -> SignalFilter/356  "<m_dot_BellValve[kg|s]>"
  BellValve/6 -> SignalFilter/357  "<Ctrl_BellValve[0_1]>"
  RearChamber/1 -> SignalFilter/358  "<m_dot_In_RearChamber[kg|s]>"
  RearChamber/2 -> SignalFilter/359  "<m_dot_Out_RearChamber[kg|s]>"
  RearChamber/3 -> SignalFilter/360  "<T_RearChamber[degC]>"
  RearChamber/4 -> SignalFilter/361  "<p_RearChamber[bar]>"
  RearChamber/5 -> SignalFilter/362  "<V_RearChamber[m3]>"
  PushRod/1 -> SignalFilter/363  "<F_Pedal[N]>"
  PushRod/2 -> SignalFilter/364  "<F_Spring[N]>"
  PushRod/3 -> SignalFilter/365  "<F_RearChamber[N]>"
  PushRod/4 -> SignalFilter/366  "<F_VacuumChamber[N]>"
  PushRod/5 -> SignalFilter/367  "<F_PushRod[N]>"
  PushRod/6 -> SignalFilter/368  "<x[m]>"
  PushRod/7 -> SignalFilter/369  "<V_delta[m3]>"
  PushRod/8 -> SignalFilter/370  "<A_Diaphragm[m2]>"
  OutputPoint/1 -> SignalFilter/371  "<F_OutputPoint[N]>"
  OutputPoint/2 -> SignalFilter/372  "<p_OutputPoint[bar]>"
  OutputPoint/3 -> SignalFilter/373  "<Pos_BrakePedal_OutputPoint[%]>"
  OutputPoint/4 -> SignalFilter/374  "<F_Max_Pedal[N]>"
  OutputPoint/5 -> SignalFilter/375  "<p_Max_Booster[bar]>"
  ControllerBellValve/1 -> SignalFilter/376  "<p_Setpoint[bar]>"
  ControllerBellValve/2 -> SignalFilter/377  "<p_MasterBrakeCyl[bar]>"
  ControllerBellValve/3 -> SignalFilter/378  "<p_delta[bar]>"
  ControllerBellValve/4 -> SignalFilter/379  "<ValveState[1ChamberCon|2AmbientCon]>"
  ControllerBellValve/5 -> SignalFilter/380  "<Ctrl_A_BellValve[0_1]>"
  ControllerBellValve/6 -> SignalFilter/381  "<F_Pedal[N]>"
  Manifold/1 -> SignalFilter/382  "<Pos_AccPedal[%]>"
  Manifold/2 -> SignalFilter/383  "<p_Manifold[bar]>"
  Position_Left/1 -> Reshape_384/1  "<Pos_Left_Wheel[x;y;z][m]>"
  Reshape_384/1 -> SignalFilter/384
  Position_Left/2 -> Reshape_385/1  "<Pos_Left_Wheel_dqL[x;y;z][]>"
  Reshape_385/1 -> SignalFilter/385
  Position_Left/3 -> Reshape_386/1  "<Pos_Left_Wheel_dqR[x;y;z][]>"
  Reshape_386/1 -> SignalFilter/386
  Position_Left/4 -> Reshape_387/1  "<Pos_Left_Wheel_dDispl_SteeringRod[x;y;z][]>"
  Reshape_387/1 -> SignalFilter/387
  Angle_Left_Wheel[Alpha;Beta;Gamma][deg]/1 -> SignalFilter/388  "<Angle_Alpha_Left_Wheel[deg]>"
  Angle_Left_Wheel[Alpha;Beta;Gamma][deg]/2 -> SignalFilter/389  "<Angle_Beta_Left_Wheel[deg]>"
  Angle_Left_Wheel[Alpha;Beta;Gamma][deg]/3 -> SignalFilter/390  "<Angle_Gamma_Left_Wheel[deg]>"
  Orientation_Left/2 -> Reshape_391/1  "<w_Rel_Left_Wheel_dqL_dt[x;y;z][rad|m]>"
  Reshape_391/1 -> SignalFilter/391
  Orientation_Left/3 -> Reshape_392/1  "<w_Rel_Left_Wheel_dqR_dt[x;y;z][rad|m]>"
  Reshape_392/1 -> SignalFilter/392
  Orientation_Left/4 -> Reshape_393/1  "<w_Rel_Left_Wheel_dDispl_SteeringRod_dt[x;y;z][rad|m]>"
  Reshape_393/1 -> SignalFilter/393
  Orientation_Left/5 -> Reshape_394/1  "<UnitVec_y_Wheel_Left_CoorSys_V[x;y;z]>"
  Reshape_394/1 -> SignalFilter/394
  Spring_Left/1 -> SignalFilter/395  "<Displ_Spring_Left[m]>"
  Spring_Left/2 -> SignalFilter/396  "<Displ_Spring_Left_dqL[]>"
  Spring_Left/3 -> SignalFilter/397  "<Displ_Spring_Left_dqR[]>"
  Damper_Left/1 -> SignalFilter/398  "<Displ_Damper_Left_dt[m|s]>"
  Damper_Left/2 -> SignalFilter/399  "<Displ_Damper_Left_dqL[]>"
  Damper_Left/3 -> SignalFilter/400  "<Displ_Damper_Left_dqR[]>"
  Damper_Left/4 -> SignalFilter/401  "<Displ_Damper_Left[m]>"
  Position_Right/1 -> Reshape_402/1  "<Pos_Right_Wheel[x;y;z][m]>"
  Reshape_402/1 -> SignalFilter/402
  Position_Right/2 -> Reshape_403/1  "<Pos_Right_Wheel_dqL[x;y;z][]>"
  Reshape_403/1 -> SignalFilter/403
  Position_Right/3 -> Reshape_404/1  "<Pos_Right_Wheel_dqR[x;y;z][]>"
  Reshape_404/1 -> SignalFilter/404
  Position_Right/4 -> Reshape_405/1  "<Pos_Right_Wheel_dDispl_SteeringRod[x;y;z][]>"
  Reshape_405/1 -> SignalFilter/405
  Angle_Right_Wheel[Alpha;Beta;Gamma][deg]/1 -> SignalFilter/406  "<Angle_Alpha_Right_Wheel[deg]>"
  Angle_Right_Wheel[Alpha;Beta;Gamma][deg]/2 -> SignalFilter/407  "<Angle_Beta_Right_Wheel[deg]>"
  Angle_Right_Wheel[Alpha;Beta;Gamma][deg]/3 -> SignalFilter/408  "<Angle_Gamma_Right_Wheel[deg]>"
  Orientation_Right/2 -> Reshape_409/1  "<w_Rel_Right_Wheel_dqL_dt[x;y;z][rad|m]>"
  Reshape_409/1 -> SignalFilter/409
  Orientation_Right/3 -> Reshape_410/1  "<w_Rel_Right_Wheel_dqR_dt[x;y;z][rad|m]>"
  Reshape_410/1 -> SignalFilter/410
  Orientation_Right/4 -> Reshape_411/1  "<w_Rel_Right_Wheel_dDispl_SteeringRod_dt[x;y;z][rad|m]>"
  Reshape_411/1 -> SignalFilter/411
  Orientation_Right/5 -> Reshape_412/1  "<UnitVec_y_Wheel_Right_CoorSys_V[x;y;z]>"
  Reshape_412/1 -> SignalFilter/412
  Spring_Right/1 -> SignalFilter/413  "<Displ_Spring_Right[m]>"
  Spring_Right/2 -> SignalFilter/414  "<Displ_Spring_Right_dqL[]>"
  Spring_Right/3 -> SignalFilter/415  "<Displ_Spring_Right_dqR[]>"
  Damper_Right/1 -> SignalFilter/416  "<Displ_Damper_Right_dt[m|s]>"
  Damper_Right/2 -> SignalFilter/417  "<Displ_Damper_Right_dqL[]>"
  Damper_Right/3 -> SignalFilter/418  "<Displ_Damper_Right_dqR[]>"
  Damper_Right/4 -> SignalFilter/419  "<Displ_Damper_Right[m]>"
  Stabilizer/1 -> SignalFilter/420  "<Displ_Stabilizer[m]>"
  Stabilizer/2 -> SignalFilter/421  "<Displ_Stabilizer_Left[m]>"
  Stabilizer/3 -> SignalFilter/422  "<Displ_Stabilizer_Right[m]>"
  Stabilizer/4 -> SignalFilter/423  "<Displ_Stabilizer_dqL[]>"
  Stabilizer/5 -> SignalFilter/424  "<Displ_Stabilizer_dqR[]>"
  SuspensionComplianceFront/1 -> Reshape_425/1  "<Angle_Comp_FR_Wheel_dt[x;y;z][rad|s]>"
  Reshape_425/1 -> SignalFilter/425
  SuspensionComplianceFront/2 -> Reshape_426/1  "<Angle_Comp_FL_Wheel_dt[x;y;z][rad|s]>"
  Reshape_426/1 -> SignalFilter/426
  SuspensionComplianceFront/3 -> Reshape_427/1  "<Angle_Comp_FR_Wheel[x;y;z][rad]>"
  Reshape_427/1 -> SignalFilter/427
  SuspensionComplianceFront/4 -> Reshape_428/1  "<Angle_Comp_FL_Wheel[x;y;z][rad]>"
  Reshape_428/1 -> SignalFilter/428
  SuspensionComplianceFront/5 -> Reshape_429/1  "<Displ_Comp_FR_Wheel_dt[x;y;z][m|s]>"
  Reshape_429/1 -> SignalFilter/429
  SuspensionComplianceFront/6 -> Reshape_430/1  "<Displ_Comp_FL_Wheel_dt[x;y;z][m|s]>"
  Reshape_430/1 -> SignalFilter/430
  SuspensionComplianceFront/7 -> Reshape_431/1  "<Displ_Comp_FR_Wheel[x;y;z][m]>"
  Reshape_431/1 -> SignalFilter/431
  SuspensionComplianceFront/8 -> Reshape_432/1  "<Displ_Comp_FL_Wheel[x;y;z][m]>"
  Reshape_432/1 -> SignalFilter/432
  ComplianceLongForce/1 -> SignalFilter/433  "<Displ_x_Wheel_F_x_Left[mm]>"
  ComplianceLongForce/2 -> SignalFilter/434  "<Displ_x_Wheel_F_x_Right[mm]>"
  ComplianceLongForce/3 -> SignalFilter/435  "<Displ_y_Wheel_F_x_Left[mm]>"
  ComplianceLongForce/4 -> SignalFilter/436  "<Displ_y_Wheel_F_x_Right[mm]>"
  ComplianceLongForce/5 -> SignalFilter/437  "<Angle_Alpha_Wheel_F_x_Left[deg]>"
  ComplianceLongForce/6 -> SignalFilter/438  "<Angle_Alpha_Wheel_F_x_Right[deg]>"
  ComplianceLongForce/7 -> SignalFilter/439  "<Angle_Gamma_Wheel_F_x_Left[deg]>"
  ComplianceLongForce/8 -> SignalFilter/440  "<Angle_Gamma_Wheel_F_x_Right[deg]>"
  ComplianceLatForce/1 -> SignalFilter/441  "<Displ_x_Wheel_F_y_Left[mm]>"
  ComplianceLatForce/2 -> SignalFilter/442  "<Displ_x_Wheel_F_y_Right[mm]>"
  ComplianceLatForce/3 -> SignalFilter/443  "<Displ_y_Wheel_F_y_Left[mm]>"
  ComplianceLatForce/4 -> SignalFilter/444  "<Displ_y_Wheel_F_y_Right[mm]>"
  ComplianceLatForce/5 -> SignalFilter/445  "<Angle_Alpha_Wheel_F_y_Left[deg]>"
  ComplianceLatForce/6 -> SignalFilter/446  "<Angle_Alpha_Wheel_F_y_Right[deg]>"
  ComplianceLatForce/7 -> SignalFilter/447  "<Angle_Gamma_Wheel_F_y_Left[deg]>"
  ComplianceLatForce/8 -> SignalFilter/448  "<Angle_Gamma_Wheel_F_y_Right[deg]>"
  ComplianceAligningTorque/1 -> SignalFilter/449  "<Displ_x_Wheel_Trq_z_Left[mm]>"
  ComplianceAligningTorque/2 -> SignalFilter/450  "<Displ_x_Wheel_Trq_z_Right[mm]>"
  ComplianceAligningTorque/3 -> SignalFilter/451  "<Displ_y_Wheel_Trq_z_Left[mm]>"
  ComplianceAligningTorque/4 -> SignalFilter/452  "<Displ_y_Wheel_Trq_z_Right[mm]>"
  ComplianceAligningTorque/5 -> SignalFilter/453  "<Angle_Alpha_Wheel_Trq_z_Left[deg]>"
  ComplianceAligningTorque/6 -> SignalFilter/454  "<Angle_Alpha_Wheel_Trq_z_Right[deg]>"
  ComplianceAligningTorque/7 -> SignalFilter/455  "<Angle_Gamma_Wheel_Trq_z_Left[deg]>"
  ComplianceAligningTorque/8 -> SignalFilter/456  "<Angle_Gamma_Wheel_Trq_z_Right[deg]>"
  ComplianceLongTorque/1 -> SignalFilter/457  "<Displ_x_Wheel_Trq_x_Left[mm]>"
  ComplianceLongTorque/2 -> SignalFilter/458  "<Displ_x_Wheel_Trq_x_Right[mm]>"
  ComplianceLongTorque/3 -> SignalFilter/459  "<Displ_y_Wheel_Trq_x_Left[mm]>"
  ComplianceLongTorque/4 -> SignalFilter/460  "<Displ_y_Wheel_Trq_x_Right[mm]>"
  ComplianceLongTorque/5 -> SignalFilter/461  "<Angle_Alpha_Wheel_Trq_x_Left[deg]>"
  ComplianceLongTorque/6 -> SignalFilter/462  "<Angle_Alpha_Wheel_Trq_x_Right[deg]>"
  ComplianceLongTorque/7 -> SignalFilter/463  "<Angle_Gamma_Wheel_Trq_x_Left[deg]>"
  ComplianceLongTorque/8 -> SignalFilter/464  "<Angle_Gamma_Wheel_Trq_x_Right[deg]>"
  SuspensionForcesFront/1 -> SignalFilter/465  "<F_FL_Spring[N]>"
  SuspensionForcesFront/2 -> SignalFilter/466  "<F_FL_Spring_dDispl_FL_Spring[N|m]>"
  SuspensionForcesFront/3 -> SignalFilter/467  "<F_FL_Damper[N]>"
  SuspensionForcesFront/4 -> SignalFilter/468  "<F_FL_Damper_dDispl_FL_Damper_dt[N|(m|s)]>"
  SuspensionForcesFront/5 -> SignalFilter/469  "<F_Stabilizer[N]>"
  SuspensionForcesFront/6 -> SignalFilter/470  "<F_Stabilizer_dDispl_Stabilizer[N|m]>"
  SuspensionForcesFront/7 -> SignalFilter/471  "<F_FR_Spring[N]>"
  SuspensionForcesFront/8 -> SignalFilter/472  "<F_FR_Spring_dDispl_FR_Spring[N|m]>"
  SuspensionForcesFront/9 -> SignalFilter/473  "<F_FR_Damper[N]>"
  SuspensionForcesFront/10 -> SignalFilter/474  "<F_FR_Damper_dDispl_FR_Damper_dt[N|(m|s)]>"
  Pos_Wheel[FL;FR][x;y;z][m]/1 -> Reshape_475/1  "<Pos_FL_Wheel[x;y;z][m]>"
  Reshape_475/1 -> SignalFilter/475
  Pos_Wheel[FL;FR][x;y;z][m]/2 -> Reshape_476/1  "<Pos_FR_Wheel[x;y;z][m]>"
  Reshape_476/1 -> SignalFilter/476
  UnitVec_y_Wheel_CoorSys_V[FL;FR][x;y;z]/1 -> Reshape_477/1  "<UnitVec_y_FL_Wheel_CoorSys_V[x;y;z]>"
  Reshape_477/1 -> SignalFilter/477
  UnitVec_y_Wheel_CoorSys_V[FL;FR][x;y;z]/2 -> Reshape_478/1  "<UnitVec_y_FR_Wheel_CoorSys_V[x;y;z]>"
  Reshape_478/1 -> SignalFilter/478
  Angle_FL_Wheel[Toe;Camber][deg]/1 -> SignalFilter/479  "<Angle_Toe_FL_Wheel_CoorSys_V[deg]>"
  Angle_FL_Wheel[Toe;Camber][deg]/2 -> SignalFilter/480  "<Angle_Camber_FL_Wheel_CoorSys_V[deg]>"
  Angle_FR_Wheel[Toe;Camber][deg]/1 -> SignalFilter/481  "<Angle_Toe_FR_Wheel_CoorSys_V[deg]>"
  Angle_FR_Wheel[Toe;Camber][deg]/2 -> SignalFilter/482  "<Angle_Camber_FR_Wheel_CoorSys_V[deg]>"
  Position_Left1/1 -> Reshape_483/1  "<Pos_Left_Wheel[x;y;z][m]>"
  Reshape_483/1 -> SignalFilter/483
  Position_Left1/2 -> Reshape_484/1  "<Pos_Left_Wheel_dqL[x;y;z][]>"
  Reshape_484/1 -> SignalFilter/484
  Position_Left1/3 -> Reshape_485/1  "<Pos_Left_Wheel_dqR[x;y;z][]>"
  Reshape_485/1 -> SignalFilter/485
  Position_Left1/4 -> Reshape_486/1  "<Pos_Left_Wheel_dDispl_SteeringRod[x;y;z][]>"
  Reshape_486/1 -> SignalFilter/486
  Angle_Left_Wheel[Alpha;Beta;Gamma][deg]1/1 -> SignalFilter/487  "<Angle_Alpha_Left_Wheel[deg]>"
  Angle_Left_Wheel[Alpha;Beta;Gamma][deg]1/2 -> SignalFilter/488  "<Angle_Beta_Left_Wheel[deg]>"
  Angle_Left_Wheel[Alpha;Beta;Gamma][deg]1/3 -> SignalFilter/489  "<Angle_Gamma_Left_Wheel[deg]>"
  Orientation_Left1/2 -> Reshape_490/1  "<w_Rel_Left_Wheel_dqL_dt[x;y;z][rad|m]>"
  Reshape_490/1 -> SignalFilter/490
  Orientation_Left1/3 -> Reshape_491/1  "<w_Rel_Left_Wheel_dqR_dt[x;y;z][rad|m]>"
  Reshape_491/1 -> SignalFilter/491
  Orientation_Left1/4 -> Reshape_492/1  "<w_Rel_Left_Wheel_dDispl_SteeringRod_dt[x;y;z][rad|m]>"
  Reshape_492/1 -> SignalFilter/492
  Orientation_Left1/5 -> Reshape_493/1  "<UnitVec_y_Wheel_Left_CoorSys_V[x;y;z]>"
  Reshape_493/1 -> SignalFilter/493
  Spring_Left1/1 -> SignalFilter/494  "<Displ_Spring_Left[m]>"
  Spring_Left1/2 -> SignalFilter/495  "<Displ_Spring_Left_dqL[]>"
  Spring_Left1/3 -> SignalFilter/496  "<Displ_Spring_Left_dqR[]>"
  Damper_Left1/1 -> SignalFilter/497  "<Displ_Damper_Left_dt[m|s]>"
  Damper_Left1/2 -> SignalFilter/498  "<Displ_Damper_Left_dqL[]>"
  Damper_Left1/3 -> SignalFilter/499  "<Displ_Damper_Left_dqR[]>"
  Damper_Left1/4 -> SignalFilter/500  "<Displ_Damper_Left[m]>"
  Position_Right1/1 -> Reshape_501/1  "<Pos_Right_Wheel[x;y;z][m]>"
  Reshape_501/1 -> SignalFilter/501
  Position_Right1/2 -> Reshape_502/1  "<Pos_Right_Wheel_dqL[x;y;z][]>"
  Reshape_502/1 -> SignalFilter/502
  Position_Right1/3 -> Reshape_503/1  "<Pos_Right_Wheel_dqR[x;y;z][]>"
  Reshape_503/1 -> SignalFilter/503
  Position_Right1/4 -> Reshape_504/1  "<Pos_Right_Wheel_dDispl_SteeringRod[x;y;z][]>"
  Reshape_504/1 -> SignalFilter/504
  Angle_Right_Wheel[Alpha;Beta;Gamma][deg]1/1 -> SignalFilter/505  "<Angle_Alpha_Right_Wheel[deg]>"
  Angle_Right_Wheel[Alpha;Beta;Gamma][deg]1/2 -> SignalFilter/506  "<Angle_Beta_Right_Wheel[deg]>"
  Angle_Right_Wheel[Alpha;Beta;Gamma][deg]1/3 -> SignalFilter/507  "<Angle_Gamma_Right_Wheel[deg]>"
  Orientation_Right1/2 -> Reshape_508/1  "<w_Rel_Right_Wheel_dqL_dt[x;y;z][rad|m]>"
  Reshape_508/1 -> SignalFilter/508
  Orientation_Right1/3 -> Reshape_509/1  "<w_Rel_Right_Wheel_dqR_dt[x;y;z][rad|m]>"
  Reshape_509/1 -> SignalFilter/509
  Orientation_Right1/4 -> Reshape_510/1  "<w_Rel_Right_Wheel_dDispl_SteeringRod_dt[x;y;z][rad|m]>"
  Reshape_510/1 -> SignalFilter/510
  Orientation_Right1/5 -> Reshape_511/1  "<UnitVec_y_Wheel_Right_CoorSys_V[x;y;z]>"
  Reshape_511/1 -> SignalFilter/511
  Spring_Right1/1 -> SignalFilter/512  "<Displ_Spring_Right[m]>"
  Spring_Right1/2 -> SignalFilter/513  "<Displ_Spring_Right_dqL[]>"
  Spring_Right1/3 -> SignalFilter/514  "<Displ_Spring_Right_dqR[]>"
  Damper_Right1/1 -> SignalFilter/515  "<Displ_Damper_Right_dt[m|s]>"
  Damper_Right1/2 -> SignalFilter/516  "<Displ_Damper_Right_dqL[]>"
  Damper_Right1/3 -> SignalFilter/517  "<Displ_Damper_Right_dqR[]>"
  Damper_Right1/4 -> SignalFilter/518  "<Displ_Damper_Right[m]>"
  Stabilizer1/1 -> SignalFilter/519  "<Displ_Stabilizer[m]>"
  Stabilizer1/2 -> SignalFilter/520  "<Displ_Stabilizer_Left[m]>"
  Stabilizer1/3 -> SignalFilter/521  "<Displ_Stabilizer_Right[m]>"
  Stabilizer1/4 -> SignalFilter/522  "<Displ_Stabilizer_dqL[]>"
  Stabilizer1/5 -> SignalFilter/523  "<Displ_Stabilizer_dqR[]>"
  SuspensionComplianceRear/1 -> Reshape_524/1  "<Angle_Comp_RR_Wheel_dt[x;y;z][rad|s]>"
  Reshape_524/1 -> SignalFilter/524
  SuspensionComplianceRear/2 -> Reshape_525/1  "<Angle_Comp_RL_Wheel_dt[x;y;z][rad|s]>"
  Reshape_525/1 -> SignalFilter/525
  SuspensionComplianceRear/3 -> Reshape_526/1  "<Angle_Comp_RR_Wheel[x;y;z][rad]>"
  Reshape_526/1 -> SignalFilter/526
  SuspensionComplianceRear/4 -> Reshape_527/1  "<Angle_Comp_RL_Wheel[x;y;z][rad]>"
  Reshape_527/1 -> SignalFilter/527
  SuspensionComplianceRear/5 -> Reshape_528/1  "<Displ_Comp_RR_Wheel_dt[x;y;z][m|s]>"
  Reshape_528/1 -> SignalFilter/528
  SuspensionComplianceRear/6 -> Reshape_529/1  "<Displ_Comp_RL_Wheel_dt[x;y;z][m|s]>"
  Reshape_529/1 -> SignalFilter/529
  SuspensionComplianceRear/7 -> Reshape_530/1  "<Displ_Comp_RR_Wheel[x;y;z][m]>"
  Reshape_530/1 -> SignalFilter/530
  SuspensionComplianceRear/8 -> Reshape_531/1  "<Displ_Comp_RL_Wheel[x;y;z][m]>"
  Reshape_531/1 -> SignalFilter/531
  ComplianceLongForce1/1 -> SignalFilter/532  "<Displ_x_Wheel_F_x_Left[mm]>"
  ComplianceLongForce1/2 -> SignalFilter/533  "<Displ_x_Wheel_F_x_Right[mm]>"
  ComplianceLongForce1/3 -> SignalFilter/534  "<Displ_y_Wheel_F_x_Left[mm]>"
  ComplianceLongForce1/4 -> SignalFilter/535  "<Displ_y_Wheel_F_x_Right[mm]>"
  ComplianceLongForce1/5 -> SignalFilter/536  "<Angle_Alpha_Wheel_F_x_Left[deg]>"
  ComplianceLongForce1/6 -> SignalFilter/537  "<Angle_Alpha_Wheel_F_x_Right[deg]>"
  ComplianceLongForce1/7 -> SignalFilter/538  "<Angle_Gamma_Wheel_F_x_Left[deg]>"
  ComplianceLongForce1/8 -> SignalFilter/539  "<Angle_Gamma_Wheel_F_x_Right[deg]>"
  ComplianceLatForce1/1 -> SignalFilter/540  "<Displ_x_Wheel_F_y_Left[mm]>"
  ComplianceLatForce1/2 -> SignalFilter/541  "<Displ_x_Wheel_F_y_Right[mm]>"
  ComplianceLatForce1/3 -> SignalFilter/542  "<Displ_y_Wheel_F_y_Left[mm]>"
  ComplianceLatForce1/4 -> SignalFilter/543  "<Displ_y_Wheel_F_y_Right[mm]>"
  ComplianceLatForce1/5 -> SignalFilter/544  "<Angle_Alpha_Wheel_F_y_Left[deg]>"
  ComplianceLatForce1/6 -> SignalFilter/545  "<Angle_Alpha_Wheel_F_y_Right[deg]>"
  ComplianceLatForce1/7 -> SignalFilter/546  "<Angle_Gamma_Wheel_F_y_Left[deg]>"
  ComplianceLatForce1/8 -> SignalFilter/547  "<Angle_Gamma_Wheel_F_y_Right[deg]>"
  ComplianceAligningTorque1/1 -> SignalFilter/548  "<Displ_x_Wheel_Trq_z_Left[mm]>"
  ComplianceAligningTorque1/2 -> SignalFilter/549  "<Displ_x_Wheel_Trq_z_Right[mm]>"
  ComplianceAligningTorque1/3 -> SignalFilter/550  "<Displ_y_Wheel_Trq_z_Left[mm]>"
  ComplianceAligningTorque1/4 -> SignalFilter/551  "<Displ_y_Wheel_Trq_z_Right[mm]>"
  ComplianceAligningTorque1/5 -> SignalFilter/552  "<Angle_Alpha_Wheel_Trq_z_Left[deg]>"
  ComplianceAligningTorque1/6 -> SignalFilter/553  "<Angle_Alpha_Wheel_Trq_z_Right[deg]>"
  ComplianceAligningTorque1/7 -> SignalFilter/554  "<Angle_Gamma_Wheel_Trq_z_Left[deg]>"
  ComplianceAligningTorque1/8 -> SignalFilter/555  "<Angle_Gamma_Wheel_Trq_z_Right[deg]>"
  ComplianceLongTorque1/1 -> SignalFilter/556  "<Displ_x_Wheel_Trq_x_Left[mm]>"
  ComplianceLongTorque1/2 -> SignalFilter/557  "<Displ_x_Wheel_Trq_x_Right[mm]>"
  ComplianceLongTorque1/3 -> SignalFilter/558  "<Displ_y_Wheel_Trq_x_Left[mm]>"
  ComplianceLongTorque1/4 -> SignalFilter/559  "<Displ_y_Wheel_Trq_x_Right[mm]>"
  ComplianceLongTorque1/5 -> SignalFilter/560  "<Angle_Alpha_Wheel_Trq_x_Left[deg]>"
  ComplianceLongTorque1/6 -> SignalFilter/561  "<Angle_Alpha_Wheel_Trq_x_Right[deg]>"
  ComplianceLongTorque1/7 -> SignalFilter/562  "<Angle_Gamma_Wheel_Trq_x_Left[deg]>"
  ComplianceLongTorque1/8 -> SignalFilter/563  "<Angle_Gamma_Wheel_Trq_x_Right[deg]>"
  SuspensionForcesRear/1 -> SignalFilter/564  "<F_RL_Spring[N]>"
  SuspensionForcesRear/2 -> SignalFilter/565  "<F_RL_Spring_dDispl_RL_Spring[N|m]>"
  SuspensionForcesRear/3 -> SignalFilter/566  "<F_RL_Damper[N]>"
  SuspensionForcesRear/4 -> SignalFilter/567  "<F_RL_Damper_dDispl_RL_Damper_dt[N|(m|s)]>"
  SuspensionForcesRear/5 -> SignalFilter/568  "<F_Stabilizer[N]>"
  SuspensionForcesRear/6 -> SignalFilter/569  "<F_Stabilizer_dDispl_Stabilizer[N|m]>"
  SuspensionForcesRear/7 -> SignalFilter/570  "<F_RR_Spring[N]>"
  SuspensionForcesRear/8 -> SignalFilter/571  "<F_RR_Spring_dDispl_RR_Spring[N|m]>"
  SuspensionForcesRear/9 -> SignalFilter/572  "<F_RR_Damper[N]>"
  SuspensionForcesRear/10 -> SignalFilter/573  "<F_RR_Damper_dDispl_RR_Damper_dt[N|(m|s)]>"
  Pos_Wheel[RL;RR][x;y;z][m]/1 -> Reshape_574/1  "<Pos_RL_Wheel[x;y;z][m]>"
  Reshape_574/1 -> SignalFilter/574
  Pos_Wheel[RL;RR][x;y;z][m]/2 -> Reshape_575/1  "<Pos_RR_Wheel[x;y;z][m]>"
  Reshape_575/1 -> SignalFilter/575
  UnitVec_y_Wheel_CoorSys_V[RL;RR][x;y;z]/1 -> Reshape_576/1  "<UnitVec_y_RL_Wheel_CoorSys_V[x;y;z]>"
  Reshape_576/1 -> SignalFilter/576
  UnitVec_y_Wheel_CoorSys_V[RL;RR][x;y;z]/2 -> Reshape_577/1  "<UnitVec_y_RR_Wheel_CoorSys_V[x;y;z]>"
  Reshape_577/1 -> SignalFilter/577
  Angle_RL_Wheel[Toe;Camber][deg]/1 -> SignalFilter/578  "<Angle_Toe_RL_Wheel_CoorSys_V[deg]>"
  Angle_RL_Wheel[Toe;Camber][deg]/2 -> SignalFilter/579  "<Angle_Camber_RL_Wheel_CoorSys_V[deg]>"
  Angle_RR_Wheel[Toe;Camber][deg]/1 -> SignalFilter/580  "<Angle_Toe_RR_Wheel_CoorSys_V[deg]>"
  Angle_RR_Wheel[Toe;Camber][deg]/2 -> SignalFilter/581  "<Angle_Camber_RR_Wheel_CoorSys_V[deg]>"
  SteeringRod_Back_Calc/1 -> SignalFilter/582  "<Sw_Backward_SteeringRod_Calc[0Off|1On]>"
  SteeringRod_Back_Calc/2 -> SignalFilter/583  "<Displ_SteeringRod[m]>"
  SteeringRod_Back_Calc/3 -> SignalFilter/584  "<Displ_SteeringRod_dt[m|s]>"
  DrivingResistances/1 -> SignalFilter/585  "<F_Driving_Res[N]>"
  SignalFilter/1 -> SignalFilterGain/1
  SignalFilterGain/1 -> MDLD_DATA_CAPTURE/1
